simulink model "rfsoc4x2_ospfb_128"  (R2021a)
(part 2 of 339)

      mask prompts: Tile224_enable "Enable Tile"; t224_enable_mts "Enable Multi-Tile Sync"; t224_sample_rate "Sampling Rate (Msps)"; t224_clk_out "Clock Out (MHz)"; t224_enable_pll "Enable Tile PLLs"; t224_ref_clk "Reference Clock (MHz)"; t224_axi_stream_clk "Required AXI4-Stream Clock (MHz)"; t224_QT_adc0_enable "Enable ADC"; t224_QT_adc0_digital_output "Digital Output Data"; t224_QT_adc0_dec_mode "Decimation Mode"; t224_QT_adc0_sample_per_cycle "Samples per AXI4-Stream Cycle"; t224_QT_adc0_mixer_type "Mixer Type"; t224_QT_adc0_mixer_mode "Mixer Mode"; t224_QT_adc0_nco_freq "NCO Frequency (GHz)"; t224_QT_adc0_nco_phase "NCO Phase"; t224_QT_adc0_coarse_freq "Frequency"; t224_QT_adc0_nyquist_zone "Nyquist Zone"; t224_QT_adc0_cal_mode "Calibration Mode"; t224_QT_adc1_enable "Enable ADC"; t224_QT_adc1_digital_output "Digital Output Data"; t224_QT_adc1_dec_mode "Decimation Mode"; t224_QT_adc1_sample_per_cycle "Samples per AXI4-Stream Cycle"; t224_QT_adc1_mixer_type "Mixer Type"; t224_QT_adc1_mixer_mode "Mixer Mode"; t224_QT_adc1_nco_freq "NCO Frequency (GHz)"; t224_QT_adc1_nco_phase "NCO Phase"; t224_QT_adc1_coarse_freq "Frequency"; t224_QT_adc1_nyquist_zone "Nyquist Zone"; t224_QT_adc1_cal_mode "Calibration Mode"; t224_QT_adc2_enable "Enable ADC"; t224_QT_adc2_digital_output "Digital Output Data"; t224_QT_adc2_dec_mode "Decimation Mode"; t224_QT_adc2_sample_per_cycle "Samples per AXI4-Stream Cycle"; t224_QT_adc2_mixer_type "Mixer Type"; t224_QT_adc2_mixer_mode "Mixer Mode"; t224_QT_adc2_nco_freq "NCO Frequency (GHz)"; t224_QT_adc2_nco_phase "NCO Phase"; t224_QT_adc2_coarse_freq "Frequency"; t224_QT_adc2_nyquist_zone "Nyquist Zone"; t224_QT_adc2_cal_mode "Calibration Mode"; t224_QT_adc3_enable "Enable ADC"; t224_QT_adc3_digital_output "Digital Output Data"; t224_QT_adc3_dec_mode "Decimation Mode"; t224_QT_adc3_sample_per_cycle "Samples per AXI4-Stream Cycle"; t224_QT_adc3_mixer_type "Mixer Type"; t224_QT_adc3_mixer_mode "Mixer Mode"; t224_QT_adc3_nco_freq "NCO Frequency (GHz)"; t224_QT_adc3_nco_phase "NCO Phase"; t224_QT_adc3_coarse_freq "Frequency"; t224_QT_adc3_nyquist_zone "Nyquist Zone"; t224_QT_adc3_cal_mode "Calibration Mode"; t224_DT_adc0_enable "Enable ADC"; t224_DT_adc0_digital_output "Digital Output Data"; t224_DT_adc0_dec_mode "Decimation Mode"; t224_DT_adc0_sample_per_cycle "Samples per AXI4-Stream Cycle"; t224_DT_adc0_mixer_type "Mixer Type"; t224_DT_adc0_mixer_mode "Mixer Mode"; t224_DT_adc0_nco_freq "NCO Frequency (GHz)"; t224_DT_adc0_nco_phase "NCO Phase"; t224_DT_adc0_coarse_freq "Frequency"; t224_DT_adc0_nyquist_zone "Nyquist Zone"; t224_DT_adc0_cal_mode "Calibration Mode"; t224_DT_adc1_enable "Enable ADC"; t224_DT_adc1_digital_output "Digital Output Data"; t224_DT_adc1_dec_mode "Decimation Mode"; t224_DT_adc1_sample_per_cycle "Samples per AXI4-Stream Cycle"; t224_DT_adc1_mixer_type "Mixer Type"; t224_DT_adc1_mixer_mode "Mixer Mode"; t224_DT_adc1_nco_freq "NCO Frequency (GHz)"; t224_DT_adc1_nco_phase "NCO Phase"; t224_DT_adc1_coarse_freq "Frequency"; t224_DT_adc1_nyquist_zone "Nyquist Zone"; t224_DT_adc1_cal_mode "Calibration Mode"; Tile225_enable "Enable Tile"; t225_enable_mts "Enable Multi-Tile Sync"; t225_sample_rate "Sampling Rate (Msps)"; t225_clk_out "Clock Out (MHz)"; t225_enable_pll "Enable Tile PLLs"; t225_ref_clk "Reference Clock (MHz)"; t225_axi_stream_clk "Required AXI4-Stream Clock (MHz)"; t225_QT_adc0_enable "Enable ADC"; t225_QT_adc0_digital_output "Digital Output Data"; t225_QT_adc0_dec_mode "Decimation Mode"; t225_QT_adc0_sample_per_cycle "Samples per AXI4-Stream Cycle"; t225_QT_adc0_mixer_type "Mixer Type"; t225_QT_adc0_mixer_mode "Mixer Mode"; t225_QT_adc0_nco_freq "NCO Frequency (GHz)"; t225_QT_adc0_nco_phase "NCO Phase"; t225_QT_adc0_coarse_freq "Frequency"; t225_QT_adc0_nyquist_zone "Nyquist Zone"; t225_QT_adc0_cal_mode "Calibration Mode"; t225_QT_adc1_enable "Enable ADC"; t225_QT_adc1_digital_output "Digital Output Data"; t225_QT_adc1_dec_mode "Decimation Mode"; t225_QT_adc1_sample_per_cycle "Samples per AXI4-Stream Cycle"; t225_QT_adc1_mixer_type "Mixer Type"; t225_QT_adc1_mixer_mode "Mixer Mode"; t225_QT_adc1_nco_freq "NCO Frequency (GHz)"; t225_QT_adc1_nco_phase "NCO Phase"; t225_QT_adc1_coarse_freq "Frequency"; t225_QT_adc1_nyquist_zone "Nyquist Zone"; t225_QT_adc1_cal_mode "Calibration Mode"; t225_QT_adc2_enable "Enable ADC"; t225_QT_adc2_digital_output "Digital Output Data"; t225_QT_adc2_dec_mode "Decimation Mode"; t225_QT_adc2_sample_per_cycle "Samples per AXI4-Stream Cycle"; t225_QT_adc2_mixer_type "Mixer Type"; t225_QT_adc2_mixer_mode "Mixer Mode"; t225_QT_adc2_nco_freq "NCO Frequency (GHz)"; t225_QT_adc2_nco_phase "NCO Phase"; t225_QT_adc2_coarse_freq "Frequency"; t225_QT_adc2_nyquist_zone "Nyquist Zone"; t225_QT_adc2_cal_mode "Calibration Mode"; t225_QT_adc3_enable "Enable ADC"; t225_QT_adc3_digital_output "Digital Output Data"; t225_QT_adc3_dec_mode "Decimation Mode"; t225_QT_adc3_sample_per_cycle "Samples per AXI4-Stream Cycle"; t225_QT_adc3_mixer_type "Mixer Type"; t225_QT_adc3_mixer_mode "Mixer Mode"; t225_QT_adc3_nco_freq "NCO Frequency (GHz)"; t225_QT_adc3_nco_phase "NCO Phase"; t225_QT_adc3_coarse_freq "Frequency"; t225_QT_adc3_nyquist_zone "Nyquist Zone"; t225_QT_adc3_cal_mode "Calibration Mode"; t225_DT_adc0_enable "Enable ADC"; t225_DT_adc0_digital_output "Digital Output Data"; t225_DT_adc0_dec_mode "Decimation Mode"; t225_DT_adc0_sample_per_cycle "Samples per AXI4-Stream Cycle"; t225_DT_adc0_mixer_type "Mixer Type"; t225_DT_adc0_mixer_mode "Mixer Mode"; t225_DT_adc0_nco_freq "NCO Frequency (GHz)"; t225_DT_adc0_nco_phase "NCO Phase"; t225_DT_adc0_coarse_freq "Frequency"; t225_DT_adc0_nyquist_zone "Nyquist Zone"; t225_DT_adc0_cal_mode "Calibration Mode"; t225_DT_adc1_enable "Enable ADC"; t225_DT_adc1_digital_output "Digital Output Data"; t225_DT_adc1_dec_mode "Decimation Mode"; t225_DT_adc1_sample_per_cycle "Samples per AXI4-Stream Cycle"; t225_DT_adc1_mixer_type "Mixer Type"; t225_DT_adc1_mixer_mode "Mixer Mode"; t225_DT_adc1_nco_freq "NCO Frequency (GHz)"; t225_DT_adc1_nco_phase "NCO Phase"; t225_DT_adc1_coarse_freq "Frequency"; t225_DT_adc1_nyquist_zone "Nyquist Zone"; t225_DT_adc1_cal_mode "Calibration Mode"; Tile226_enable "Enable Tile"; t226_enable_mts "Enable Multi-Tile Sync"; t226_sample_rate "Sampling Rate (Msps)"; t226_clk_out "Clock Out (MHz)"; t226_enable_pll "Enable Tile PLLs"; t226_ref_clk "Reference Clock (MHz)"; t226_axi_stream_clk "Required AXI4-Stream Clock (MHz)"; t226_QT_adc0_enable "Enable ADC"; t226_QT_adc0_digital_output "Digital Output Data"; t226_QT_adc0_dec_mode "Decimation Mode"; t226_QT_adc0_sample_per_cycle "Samples per AXI4-Stream Cycle"; t226_QT_adc0_mixer_type "Mixer Type"; t226_QT_adc0_mixer_mode "Mixer Mode"; t226_QT_adc0_nco_freq "NCO Frequency (GHz)"; t226_QT_adc0_nco_phase "NCO Phase"; t226_QT_adc0_coarse_freq "Frequency"; t226_QT_adc0_nyquist_zone "Nyquist Zone"; t226_QT_adc0_cal_mode "Calibration Mode"; t226_QT_adc1_enable "Enable ADC"; t226_QT_adc1_digital_output "Digital Output Data"; t226_QT_adc1_dec_mode "Decimation Mode"; t226_QT_adc1_sample_per_cycle "Samples per AXI4-Stream Cycle"; t226_QT_adc1_mixer_type "Mixer Type"; t226_QT_adc1_mixer_mode "Mixer Mode"; t226_QT_adc1_nco_freq "NCO Frequency (GHz)"; t226_QT_adc1_nco_phase "NCO Phase"; t226_QT_adc1_coarse_freq "Frequency"; t226_QT_adc1_nyquist_zone "Nyquist Zone"; t226_QT_adc1_cal_mode "Calibration Mode"; t226_QT_adc2_enable "Enable ADC"; t226_QT_adc2_digital_output "Digital Output Data"; t226_QT_adc2_dec_mode "Decimation Mode"; t226_QT_adc2_sample_per_cycle "Samples per AXI4-Stream Cycle"; t226_QT_adc2_mixer_type "Mixer Type"; t226_QT_adc2_mixer_mode "Mixer Mode"; t226_QT_adc2_nco_freq "NCO Frequency (GHz)"; t226_QT_adc2_nco_phase "NCO Phase"; t226_QT_adc2_coarse_freq "Frequency"; t226_QT_adc2_nyquist_zone "Nyquist Zone"; t226_QT_adc2_cal_mode "Calibration Mode"; t226_QT_adc3_enable "Enable ADC"; t226_QT_adc3_digital_output "Digital Output Data"; t226_QT_adc3_dec_mode "Decimation Mode"; t226_QT_adc3_sample_per_cycle "Samples per AXI4-Stream Cycle"; t226_QT_adc3_mixer_type "Mixer Type"; t226_QT_adc3_mixer_mode "Mixer Mode"; t226_QT_adc3_nco_freq "NCO Frequency (GHz)"; t226_QT_adc3_nco_phase "NCO Phase"; t226_QT_adc3_coarse_freq "Frequency"; t226_QT_adc3_nyquist_zone "Nyquist Zone"; t226_QT_adc3_cal_mode "Calibration Mode"; t226_DT_adc0_enable "Enable ADC"; t226_DT_adc0_digital_output "Digital Output Data"; t226_DT_adc0_dec_mode "Decimation Mode"; t226_DT_adc0_sample_per_cycle "Samples per AXI4-Stream Cycle"; t226_DT_adc0_mixer_type "Mixer Type"; t226_DT_adc0_mixer_mode "Mixer Mode"; t226_DT_adc0_nco_freq "NCO Frequency (GHz)"; t226_DT_adc0_nco_phase "NCO Phase"; t226_DT_adc0_coarse_freq "Frequency"; t226_DT_adc0_nyquist_zone "Nyquist Zone"; t226_DT_adc0_cal_mode "Calibration Mode"; t226_DT_adc1_enable "Enable ADC"; t226_DT_adc1_digital_output "Digital Output Data"; t226_DT_adc1_dec_mode "Decimation Mode"; t226_DT_adc1_sample_per_cycle "Samples per AXI4-Stream Cycle"; t226_DT_adc1_mixer_type "Mixer Type"; t226_DT_adc1_mixer_mode "Mixer Mode"; t226_DT_adc1_nco_freq "NCO Frequency (GHz)"; t226_DT_adc1_nco_phase "NCO Phase"; t226_DT_adc1_coarse_freq "Frequency"; t226_DT_adc1_nyquist_zone "Nyquist Zone"; t226_DT_adc1_cal_mode "Calibration Mode"; Tile227_enable "Enable Tile"; t227_enable_mts "Enable Multi-Tile Sync"; t227_sample_rate "Sampling Rate (Msps)"; t227_clk_out "Clock Out (MHz)"; t227_enable_pll "Enable Tile PLLs"; t227_ref_clk "Reference Clock (MHz)"; t227_axi_stream_clk "Required AXI4-Stream Clock (MHz)"; t227_QT_adc0_enable "Enable ADC"; t227_QT_adc0_digital_output "Digital Output Data"; t227_QT_adc0_dec_mode "Decimation Mode"; t227_QT_adc0_sample_per_cycle "Samples per AXI4-Stream Cycle"; t227_QT_adc0_mixer_type "Mixer Type"; t227_QT_adc0_mixer_mode "Mixer Mode"; t227_QT_adc0_nco_freq "NCO Frequency (GHz)"; t227_QT_adc0_nco_phase "NCO Phase"; t227_QT_adc0_coarse_freq "Frequency"; t227_QT_adc0_nyquist_zone "Nyquist Zone"; t227_QT_adc0_cal_mode "Calibration Mode"; t227_QT_adc1_enable "Enable ADC"; t227_QT_adc1_digital_output "Digital Output Data"; t227_QT_adc1_dec_mode "Decimation Mode"; t227_QT_adc1_sample_per_cycle "Samples per AXI4-Stream Cycle"; t227_QT_adc1_mixer_type "Mixer Type"; t227_QT_adc1_mixer_mode "Mixer Mode"; t227_QT_adc1_nco_freq "NCO Frequency (GHz)"; t227_QT_adc1_nco_phase "NCO Phase"; t227_QT_adc1_coarse_freq "Frequency"; t227_QT_adc1_nyquist_zone "Nyquist Zone"; t227_QT_adc1_cal_mode "Calibration Mode"; t227_QT_adc2_enable "Enable ADC"; t227_QT_adc2_digital_output "Digital Output Data"; t227_QT_adc2_dec_mode "Decimation Mode"; t227_QT_adc2_sample_per_cycle "Samples per AXI4-Stream Cycle"; t227_QT_adc2_mixer_type "Mixer Type"; t227_QT_adc2_mixer_mode "Mixer Mode"; t227_QT_adc2_nco_freq "NCO Frequency (GHz)"; t227_QT_adc2_nco_phase "NCO Phase"; t227_QT_adc2_coarse_freq "Frequency"; t227_QT_adc2_nyquist_zone "Nyquist Zone"; t227_QT_adc2_cal_mode "Calibration Mode"; t227_QT_adc3_enable "Enable ADC"; t227_QT_adc3_digital_output "Digital Output Data"; t227_QT_adc3_dec_mode "Decimation Mode"; t227_QT_adc3_sample_per_cycle "Samples per AXI4-Stream Cycle"; t227_QT_adc3_mixer_type "Mixer Type"; t227_QT_adc3_mixer_mode "Mixer Mode"; t227_QT_adc3_nco_freq "NCO Frequency (GHz)"; t227_QT_adc3_nco_phase "NCO Phase"; t227_QT_adc3_coarse_freq "Frequency"; t227_QT_adc3_nyquist_zone "Nyquist Zone"; t227_QT_adc3_cal_mode "Calibration Mode"; t227_DT_adc0_enable "Enable ADC"; t227_DT_adc0_digital_output "Digital Output Data"; t227_DT_adc0_dec_mode "Decimation Mode"; t227_DT_adc0_sample_per_cycle "Samples per AXI4-Stream Cycle"; t227_DT_adc0_mixer_type "Mixer Type"; t227_DT_adc0_mixer_mode "Mixer Mode"; t227_DT_adc0_nco_freq "NCO Frequency (GHz)"; t227_DT_adc0_nco_phase "NCO Phase"; t227_DT_adc0_coarse_freq "Frequency"; t227_DT_adc0_nyquist_zone "Nyquist Zone"; t227_DT_adc0_cal_mode "Calibration Mode"; t227_DT_adc1_enable "Enable ADC"; t227_DT_adc1_digital_output "Digital Output Data"; t227_DT_adc1_dec_mode "Decimation Mode"; t227_DT_adc1_sample_per_cycle "Samples per AXI4-Stream Cycle"; t227_DT_adc1_mixer_type "Mixer Type"; t227_DT_adc1_mixer_mode "Mixer Mode"; t227_DT_adc1_nco_freq "NCO Frequency (GHz)"; t227_DT_adc1_nco_phase "NCO Phase"; t227_DT_adc1_coarse_freq "Frequency"; t227_DT_adc1_nyquist_zone "Nyquist Zone"; t227_DT_adc1_cal_mode "Calibration Mode"; Tile228_enable "Enable Tile"; t228_enable_mts "Enable Multi-Tile Sync"; t228_sample_rate "Sampling Rate (Msps)"; t228_clk_out "Clock Out (MHz)"; t228_enable_pll "Enable Tile PLLs"; t228_ref_clk "Reference Clock (MHz)"; t228_axi_stream_clk "Required AXI4-Stream Clock (MHz)"; t228_output_power "Output Power"; t228_QT_dac0_enable "Enable DAC"; t228_QT_dac0_analog_output "Analog Output Data"; t228_QT_dac0_inter_mode "Interpolation Mode"; t228_QT_dac0_sample_per_cycle "Samples per AXI4-Stream Cycle"; t228_QT_dac0_datapath_mode "Datapath Mode"; t228_QT_dac0_mixer_type "Mixer Type"; t228_QT_dac0_mixer_mode "Mixer Mode"; t228_QT_dac0_nco_freq "NCO Frequency (GHz)"; t228_QT_dac0_nco_phase "NCO Phase"; t228_QT_dac0_coarse_freq "Frequency"; t228_QT_dac0_nyquist_zone "Nyquist Zone"; t228_QT_dac0_decode_mode "Decoder Mode"; t228_QT_dac1_enable "Enable DAC"; t228_QT_dac1_analog_output "Analog Output Data"; t228_QT_dac1_inter_mode "Interpolation Mode"; t228_QT_dac1_sample_per_cycle "Samples per AXI4-Stream Cycle"; t228_QT_dac1_datapath_mode "Datapath Mode"; t228_QT_dac1_mixer_type "Mixer Type"; t228_QT_dac1_mixer_mode "Mixer Mode"; t228_QT_dac1_nco_freq "NCO Frequency (GHz)"; t228_QT_dac1_nco_phase "NCO Phase"; t228_QT_dac1_coarse_freq "Frequency"; t228_QT_dac1_nyquist_zone "Nyquist Zone"; t228_QT_dac1_decode_mode "Decoder Mode"; t228_QT_dac2_enable "Enable DAC"; t228_QT_dac2_analog_output "Analog Output Data"; t228_QT_dac2_inter_mode "Interpolation Mode"; t228_QT_dac2_sample_per_cycle "Samples per AXI4-Stream Cycle"; t228_QT_dac2_datapath_mode "Datapath Mode"; t228_QT_dac2_mixer_type "Mixer Type"; t228_QT_dac2_mixer_mode "Mixer Mode"; t228_QT_dac2_nco_freq "NCO Frequency (GHz)"; t228_QT_dac2_nco_phase "NCO Phase"; t228_QT_dac2_coarse_freq "Frequency"; t228_QT_dac2_nyquist_zone "Nyquist Zone"; t228_QT_dac2_decode_mode "Decoder Mode"; t228_QT_dac3_enable "Enable DAC"; t228_QT_dac3_analog_output "Analog Output Data"; t228_QT_dac3_inter_mode "Interpolation Mode"; t228_QT_dac3_sample_per_cycle "Samples per AXI4-Stream Cycle"; t228_QT_dac3_datapath_mode "Datapath Mode"; t228_QT_dac3_mixer_type "Mixer Type"; t228_QT_dac3_mixer_mode "Mixer Mode"; t228_QT_dac3_nco_freq "NCO Frequency (GHz)"; t228_QT_dac3_nco_phase "NCO Phase"; t228_QT_dac3_coarse_freq "Frequency"; t228_QT_dac3_nyquist_zone "Nyquist Zone"; t228_QT_dac3_decode_mode "Decoder Mode"; t228_DT_dac0_enable "Enable DAC"; t228_DT_dac0_analog_output "Analog Output Data"; t228_DT_dac0_inter_mode "Interpolation Mode"; t228_DT_dac0_sample_per_cycle "Samples per AXI4-Stream Cycle"; t228_DT_dac0_mixer_type "Mixer Type"; t228_DT_dac0_mixer_mode "Mixer Mode"; t228_DT_dac0_nco_freq "NCO Frequency (GHz)"; t228_DT_dac0_nco_phase "NCO Phase"; t228_DT_dac0_coarse_freq "Frequency"; t228_DT_dac0_nyquist_zone "Nyquist Zone"; t228_DT_dac0_decode_mode "Decoder Mode"; t228_DT_dac1_enable "Enable DAC"; t228_DT_dac1_analog_output "Analog Output Data"; t228_DT_dac1_inter_mode "Interpolation Mode"; t228_DT_dac1_sample_per_cycle "Samples per AXI4-Stream Cycle"; t228_DT_dac1_mixer_type "Mixer Type"; t228_DT_dac1_mixer_mode "Mixer Mode"; t228_DT_dac1_nco_freq "NCO Frequency (GHz)"; t228_DT_dac1_nco_phase "NCO Phase"; t228_DT_dac1_coarse_freq "Frequency"; t228_DT_dac1_nyquist_zone "Nyquist Zone"; t228_DT_dac1_decode_mode "Decoder Mode"; Tile229_enable "Enable Tile"; t229_enable_mts "Enable Multi-Tile Sync"; t229_sample_rate "Sampling Rate (Msps)"; t229_clk_out "Clock Out (MHz)"; t229_enable_pll "Enable Tile PLLs"; t229_ref_clk "Reference Clock (MHz)"; t229_axi_stream_clk "Required AXI4-Stream Clock (MHz)"; t229_output_power "Output Power"; t229_QT_dac0_enable "Enable DAC"; t229_QT_dac0_analog_output "Analog Output Data"; t229_QT_dac0_inter_mode "Interpolation Mode"; t229_QT_dac0_sample_per_cycle "Samples per AXI4-Stream Cycle"; t229_QT_dac0_datapath_mode "Datapath Mode"; t229_QT_dac0_mixer_type "Mixer Type"; t229_QT_dac0_mixer_mode "Mixer Mode"; t229_QT_dac0_nco_freq "NCO Frequency (GHz)"; t229_QT_dac0_nco_phase "NCO Phase"; t229_QT_dac0_coarse_freq "Frequency"; t229_QT_dac0_nyquist_zone "Nyquist Zone"; t229_QT_dac0_decode_mode "Decoder Mode"; t229_QT_dac1_enable "Enable DAC"; t229_QT_dac1_analog_output "Analog Output Data"; t229_QT_dac1_inter_mode "Interpolation Mode"; t229_QT_dac1_sample_per_cycle "Samples per AXI4-Stream Cycle"; t229_QT_dac1_datapath_mode "Datapath Mode"; t229_QT_dac1_mixer_type "Mixer Type"; t229_QT_dac1_mixer_mode "Mixer Mode"; t229_QT_dac1_nco_freq "NCO Frequency (GHz)"; t229_QT_dac1_nco_phase "NCO Phase"; t229_QT_dac1_coarse_freq "Frequency"; t229_QT_dac1_nyquist_zone "Nyquist Zone"; t229_QT_dac1_decode_mode "Decoder Mode"; t229_QT_dac2_enable "Enable DAC"; t229_QT_dac2_analog_output "Analog Output Data"; t229_QT_dac2_inter_mode "Interpolation Mode"; t229_QT_dac2_sample_per_cycle "Samples per AXI4-Stream Cycle"; t229_QT_dac2_datapath_mode "Datapath Mode"; t229_QT_dac2_mixer_type "Mixer Type"; t229_QT_dac2_mixer_mode "Mixer Mode"; t229_QT_dac2_nco_freq "NCO Frequency (GHz)"; t229_QT_dac2_nco_phase "NCO Phase"; t229_QT_dac2_coarse_freq "Frequency"; t229_QT_dac2_nyquist_zone "Nyquist Zone"; t229_QT_dac2_decode_mode "Decoder Mode"; t229_QT_dac3_enable "Enable DAC"; t229_QT_dac3_analog_output "Analog Output Data"; t229_QT_dac3_inter_mode "Interpolation Mode"; t229_QT_dac3_sample_per_cycle "Samples per AXI4-Stream Cycle"; t229_QT_dac3_datapath_mode "Datapath Mode"; t229_QT_dac3_mixer_type "Mixer Type"; t229_QT_dac3_mixer_mode "Mixer Mode"; t229_QT_dac3_nco_freq "NCO Frequency (GHz)"; t229_QT_dac3_nco_phase "NCO Phase"; t229_QT_dac3_coarse_freq "Frequency"; t229_QT_dac3_nyquist_zone "Nyquist Zone"; t229_QT_dac3_decode_mode "Decoder Mode"; t229_DT_dac0_enable "Enable DAC"; t229_DT_dac0_analog_output "Analog Output Data"; t229_DT_dac0_inter_mode "Interpolation Mode"; t229_DT_dac0_sample_per_cycle "Samples per AXI4-Stream Cycle"; t229_DT_dac0_mixer_type "Mixer Type"; t229_DT_dac0_mixer_mode "Mixer Mode"; t229_DT_dac0_nco_freq "NCO Frequency (GHz)"; t229_DT_dac0_nco_phase "NCO Phase"; t229_DT_dac0_coarse_freq "Frequency"; t229_DT_dac0_nyquist_zone "Nyquist Zone"; t229_DT_dac0_decode_mode "Decoder Mode"; t229_DT_dac1_enable "Enable DAC"; t229_DT_dac1_analog_output "Analog Output Data"; t229_DT_dac1_inter_mode "Interpolation Mode"; t229_DT_dac1_sample_per_cycle "Samples per AXI4-Stream Cycle"; t229_DT_dac1_mixer_type "Mixer Type"; t229_DT_dac1_mixer_mode "Mixer Mode"; t229_DT_dac1_nco_freq "NCO Frequency (GHz)"; t229_DT_dac1_nco_phase "NCO Phase"; t229_DT_dac1_coarse_freq "Frequency"; t229_DT_dac1_nyquist_zone "Nyquist Zone"; t229_DT_dac1_decode_mode "Decoder Mode"; Tile230_enable "Enable Tile"; t230_enable_mts "Enable Multi-Tile Sync"; t230_sample_rate "Sampling Rate (Msps)"; t230_clk_out "Clock Out (MHz)"; t230_enable_pll "Enable Tile PLLs"; t230_ref_clk "Reference Clock (MHz)"; t230_axi_stream_clk "Required AXI4-Stream Clock (MHz)"; t230_output_power "Output Power"; t230_QT_dac0_enable "Enable DAC"; t230_QT_dac0_analog_output "Analog Output Data"; t230_QT_dac0_inter_mode "Interpolation Mode"; t230_QT_dac0_sample_per_cycle "Samples per AXI4-Stream Cycle"; t230_QT_dac0_datapath_mode "Datapath Mode"; t230_QT_dac0_mixer_type "Mixer Type"; t230_QT_dac0_mixer_mode "Mixer Mode"; t230_QT_dac0_nco_freq "NCO Frequency (GHz)"; t230_QT_dac0_nco_phase "NCO Phase"; t230_QT_dac0_coarse_freq "Frequency"; t230_QT_dac0_nyquist_zone "Nyquist Zone"; t230_QT_dac0_decode_mode "Decoder Mode"; t230_QT_dac1_enable "Enable DAC"; t230_QT_dac1_analog_output "Analog Output Data"; t230_QT_dac1_inter_mode "Interpolation Mode"; t230_QT_dac1_sample_per_cycle "Samples per AXI4-Stream Cycle"; t230_QT_dac1_datapath_mode "Datapath Mode"; t230_QT_dac1_mixer_type "Mixer Type"; t230_QT_dac1_mixer_mode "Mixer Mode"; t230_QT_dac1_nco_freq "NCO Frequency (GHz)"; t230_QT_dac1_nco_phase "NCO Phase"; t230_QT_dac1_coarse_freq "Frequency"; t230_QT_dac1_nyquist_zone "Nyquist Zone"; t230_QT_dac1_decode_mode "Decoder Mode"; t230_QT_dac2_enable "Enable DAC"; t230_QT_dac2_analog_output "Analog Output Data"; t230_QT_dac2_inter_mode "Interpolation Mode"; t230_QT_dac2_sample_per_cycle "Samples per AXI4-Stream Cycle"; t230_QT_dac2_datapath_mode "Datapath Mode"; t230_QT_dac2_mixer_type "Mixer Type"; t230_QT_dac2_mixer_mode "Mixer Mode"; t230_QT_dac2_nco_freq "NCO Frequency (GHz)"; t230_QT_dac2_nco_phase "NCO Phase"; t230_QT_dac2_coarse_freq "Frequency"; t230_QT_dac2_nyquist_zone "Nyquist Zone"; t230_QT_dac2_decode_mode "Decoder Mode"; t230_QT_dac3_enable "Enable DAC"; t230_QT_dac3_analog_output "Analog Output Data"; t230_QT_dac3_inter_mode "Interpolation Mode"; t230_QT_dac3_sample_per_cycle "Samples per AXI4-Stream Cycle"; t230_QT_dac3_datapath_mode "Datapath Mode"; t230_QT_dac3_mixer_type "Mixer Type"; t230_QT_dac3_mixer_mode "Mixer Mode"; t230_QT_dac3_nco_freq "NCO Frequency (GHz)"; t230_QT_dac3_nco_phase "NCO Phase"; t230_QT_dac3_coarse_freq "Frequency"; t230_QT_dac3_nyquist_zone "Nyquist Zone"; t230_QT_dac3_decode_mode "Decoder Mode"; t230_DT_dac0_enable "Enable DAC"; t230_DT_dac0_analog_output "Analog Output Data"; t230_DT_dac0_inter_mode "Interpolation Mode"; t230_DT_dac0_sample_per_cycle "Samples per AXI4-Stream Cycle"; t230_DT_dac0_mixer_type "Mixer Type"; t230_DT_dac0_mixer_mode "Mixer Mode"; t230_DT_dac0_nco_freq "NCO Frequency (GHz)"; t230_DT_dac0_nco_phase "NCO Phase"; t230_DT_dac0_coarse_freq "Frequency"; t230_DT_dac0_nyquist_zone "Nyquist Zone"; t230_DT_dac0_decode_mode "Decoder Mode"; t230_DT_dac1_enable "Enable DAC"; t230_DT_dac1_analog_output "Analog Output Data"; t230_DT_dac1_inter_mode "Interpolation Mode"; t230_DT_dac1_sample_per_cycle "Samples per AXI4-Stream Cycle"; t230_DT_dac1_mixer_type "Mixer Type"; t230_DT_dac1_mixer_mode "Mixer Mode"; t230_DT_dac1_nco_freq "NCO Frequency (GHz)"; t230_DT_dac1_nco_phase "NCO Phase"; t230_DT_dac1_coarse_freq "Frequency"; t230_DT_dac1_nyquist_zone "Nyquist Zone"; t230_DT_dac1_decode_mode "Decoder Mode"; Tile231_enable "Enable Tile"; t231_enable_mts "Enable Multi-Tile Sync"; t231_sample_rate "Sampling Rate (Msps)"; t231_clk_out "Clock Out (MHz)"; t231_enable_pll "Enable Tile PLLs"; t231_ref_clk "Reference Clock (MHz)"; t231_axi_stream_clk "Required AXI4-Stream Clock (MHz)"; t231_output_power "Output Power"; t231_QT_dac0_enable "Enable DAC"; t231_QT_dac0_analog_output "Analog Output Data"; t231_QT_dac0_inter_mode "Interpolation Mode"; t231_QT_dac0_sample_per_cycle "Samples per AXI4-Stream Cycle"; t231_QT_dac0_datapath_mode "Datapath Mode"; t231_QT_dac0_mixer_type "Mixer Type"; t231_QT_dac0_mixer_mode "Mixer Mode"; t231_QT_dac0_nco_freq "NCO Frequency (GHz)"; t231_QT_dac0_nco_phase "NCO Phase"; t231_QT_dac0_coarse_freq "Frequency"; t231_QT_dac0_nyquist_zone "Nyquist Zone"; t231_QT_dac0_decode_mode "Decoder Mode"; t231_QT_dac1_enable "Enable DAC"; t231_QT_dac1_analog_output "Analog Output Data"; t231_QT_dac1_inter_mode "Interpolation Mode"; t231_QT_dac1_sample_per_cycle "Samples per AXI4-Stream Cycle"; t231_QT_dac1_datapath_mode "Datapath Mode"; t231_QT_dac1_mixer_type "Mixer Type"; t231_QT_dac1_mixer_mode "Mixer Mode"; t231_QT_dac1_nco_freq "NCO Frequency (GHz)"; t231_QT_dac1_nco_phase "NCO Phase"; t231_QT_dac1_coarse_freq "Frequency"; t231_QT_dac1_nyquist_zone "Nyquist Zone"; t231_QT_dac1_decode_mode "Decoder Mode"; t231_QT_dac2_enable "Enable DAC"; t231_QT_dac2_analog_output "Analog Output Data"; t231_QT_dac2_inter_mode "Interpolation Mode"; t231_QT_dac2_sample_per_cycle "Samples per AXI4-Stream Cycle"; t231_QT_dac2_datapath_mode "Datapath Mode"; t231_QT_dac2_mixer_type "Mixer Type"; t231_QT_dac2_mixer_mode "Mixer Mode"; t231_QT_dac2_nco_freq "NCO Frequency (GHz)"; t231_QT_dac2_nco_phase "NCO Phase"; t231_QT_dac2_coarse_freq "Frequency"; t231_QT_dac2_nyquist_zone "Nyquist Zone"; t231_QT_dac2_decode_mode "Decoder Mode"; t231_QT_dac3_enable "Enable DAC"; t231_QT_dac3_analog_output "Analog Output Data"; t231_QT_dac3_inter_mode "Interpolation Mode"; t231_QT_dac3_sample_per_cycle "Samples per AXI4-Stream Cycle"; t231_QT_dac3_datapath_mode "Datapath Mode"; t231_QT_dac3_mixer_type "Mixer Type"; t231_QT_dac3_mixer_mode "Mixer Mode"; t231_QT_dac3_nco_freq "NCO Frequency (GHz)"; t231_QT_dac3_nco_phase "NCO Phase"; t231_QT_dac3_coarse_freq "Frequency"; t231_QT_dac3_nyquist_zone "Nyquist Zone"; t231_QT_dac3_decode_mode "Decoder Mode"; t231_DT_dac0_enable "Enable DAC"; t231_DT_dac0_analog_output "Analog Output Data"; t231_DT_dac0_inter_mode "Interpolation Mode"; t231_DT_dac0_sample_per_cycle "Samples per AXI4-Stream Cycle"; t231_DT_dac0_mixer_type "Mixer Type"; t231_DT_dac0_mixer_mode "Mixer Mode"; t231_DT_dac0_nco_freq "NCO Frequency (GHz)"; t231_DT_dac0_nco_phase "NCO Phase"; t231_DT_dac0_coarse_freq "Frequency"; t231_DT_dac0_nyquist_zone "Nyquist Zone"; t231_DT_dac0_decode_mode "Decoder Mode"; t231_DT_dac1_enable "Enable DAC"; t231_DT_dac1_analog_output "Analog Output Data"; t231_DT_dac1_inter_mode "Interpolation Mode"; t231_DT_dac1_sample_per_cycle "Samples per AXI4-Stream Cycle"; t231_DT_dac1_mixer_type "Mixer Type"; t231_DT_dac1_mixer_mode "Mixer Mode"; t231_DT_dac1_nco_freq "NCO Frequency (GHz)"; t231_DT_dac1_nco_phase "NCO Phase"; t231_DT_dac1_coarse_freq "Frequency"; t231_DT_dac1_nyquist_zone "Nyquist Zone"; t231_DT_dac1_decode_mode "Decoder Mode"; t224_has_adc_clk "Has Clock"; t224_adc_clk_src "Clock Source Tile"; t224_clk_dist "Distribute Clock"; t225_has_adc_clk "Has Clock"; t225_adc_clk_src "Clock Source Tile"; t225_clk_dist "Distribute Clock"; t226_has_adc_clk "Has Clock"; t226_adc_clk_src "Clock Source Tile"; t226_clk_dist "Distribute Clock"; t227_has_adc_clk "Has Clock"; t227_adc_clk_src "Clock Source Tile"; t227_clk_dist "Distribute Clock"; t228_has_dac_clk "Has Clock"; t228_dac_clk_src "Clock Source Tile"; t228_clk_dist "Distribute Clock"; t229_has_dac_clk "Has Clock"; t229_dac_clk_src "Clock Source Tile"; t229_clk_dist "Distribute Clock"; t230_has_dac_clk "Has Clock"; t230_dac_clk_src "Clock Source Tile"; t230_clk_dist "Distribute Clock"; t231_has_dac_clk "Has Clock"; t231_dac_clk_src "Clock Source Tile"; t231_clk_dist "Distribute Clock"
      mask help: CASPER RFDC
      mask init:
      | if chk_param(gcb,'runinit','1')
      |     if chk_param(gcb,'forceredraw','0')
      |         rfdc_mask(gcb,0);
      |     else
      |         rfdc_mask(gcb,1);
      |         set_param(gcb,'forceredraw','0')
      |     end
      |     if chk_param(gcb,'maskopening','1')
      |         set_param(gcb,'runinit','0')
      |     end
      | end
      mask Help: eval('xlWeb([getenv(''MLIB_ROOT''), ''\doc\html\adc_zcu111\adc_zcu111.html''])')
      mask Callback maskopening:
      | %assignin('base','mask_opening',1)
      | %assignin('base','run_init',1)
      | set_param(gcb,'maskopening','1')
      mask Callback runinit: set_param(gcb,'runinit','1')
      mask Callback Tile224_enable: enable_mts_opt(gcb);
      mask Callback t224_sample_rate: update_rfdc_clocking(gcb,224);
      mask TypeOptions t224_clk_out: 150 | 75 | 37.5 | 18.75
      mask Callback t224_enable_pll:
      | %update_rfdc_clocking(gcb);
      | update_pll(gcb,224);
      mask TypeOptions t224_ref_clk: 738.462 | 685.714 | 640 | 600 | 564.706 | 533.333 | 505.263 | 480 | 457.143 | 436.364 | 417.391 | 400 | 384 | 369.231 | 355.556 | 342.857 | 331.034 | 320 | 309.677 | 300 | 290.909 | 282.353 | 274.286 | 266.667 | 259.459 | 252.632 | 246.154 | 240 | 234.146 | 228.571 | 223.256 | 218.182 | 213.333 | 208.696 | 204.255 | 200 | 195.918 | 192 | 188.235 | 184.615 | 181.132 | 177.778 | 174.545 | 171.429 | 168.421 | 165.517 | 162.712 | 160 | 157.377 | 154.839 | 152.381 | 150 | 147.692 | 145.455 | 143.284 | 141.176 | 139.13 | 137.143 | 135.211 | 133.333 | 131.507 | 129.73 | 128 | 126.316 | 124.675 | 123.077 | 121.519 | 120 | 118.519 | 117.073 | 115.663 | 114.286 | 112.941 | 111.628 | 110.345 | 109.091 | 107.865 | 106.667 | 105.495 | 104.348 | 103.226
      mask Callback t224_QT_adc0_enable: enable_adc_opt(gcb,224,0,'QT');
      mask TypeOptions t224_QT_adc0_digital_output: Real | I/Q
      mask Callback t224_QT_adc0_digital_output:
      | validate_digital_data(gcb,224,0,'QT');
      | update_axis_clk(gcb,224);
      mask TypeOptions t224_QT_adc0_dec_mode: 1x | 2x | 3x | 4x | 5x | 6x | 8x | 10x | 12x | 16x | 20x | 24x | 40x
      mask Callback t224_QT_adc0_dec_mode:
      | % if I/Q output mode, need to copy interp factor before updating axis clk
      | % note only the even slice for the tile makes this check
      | if chk_param(gcb, 't224_QT_adc0_mixer_mode', 'I/Q -> I/Q')
      |   dec_mode = get_param(gcb, 't224_QT_adc0_dec_mode');
      |   set_param(gcb, 't224_QT_adc1_dec_mode', dec_mode);
      | end
      | 
      | update_axis_clk(gcb,224);
      mask TypeOptions t224_QT_adc0_sample_per_cycle: 4 | 5 | 6 | 7 | 8 | 9 | 10 | 11 | 12
      mask Callback t224_QT_adc0_sample_per_cycle:
      | % if I/Q output mode, need to copy samples per clk before updating axis clk
      | % note only the even slice for the tile makes this check
      | if chk_param(gcb, 't224_QT_adc0_mixer_mode', 'I/Q -> I/Q')
      |   spc = get_param(gcb, 't224_QT_adc0_sample_per_cycle');
      |   set_param(gcb, 't224_QT_adc1_sample_per_cycle', spc);
      | end
      | update_axis_clk_label(gcb,224);
      mask TypeOptions t224_QT_adc0_mixer_type: Bypassed
      mask Callback t224_QT_adc0_mixer_type: mixertype_callback(gcb,224,0,'QT');
      mask TypeOptions t224_QT_adc0_mixer_mode: Real -> Real
      mask Callback t224_QT_adc0_mixer_mode: mixer_callback(gcb,224,0,'QT');
      mask TypeOptions t224_QT_adc0_coarse_freq: 0
      mask TypeOptions t224_QT_adc0_nyquist_zone: Zone 1 | Zone 2
      mask TypeOptions t224_QT_adc0_cal_mode: Mode 1 | Mode 2
      mask Callback t224_QT_adc1_enable: enable_adc_opt(gcb,224,1,'QT');
      mask TypeOptions t224_QT_adc1_digital_output: Real | I/Q
      mask Callback t224_QT_adc1_digital_output:
      | validate_digital_data(gcb,224,1,'QT');
      | update_axis_clk(gcb,224);
      mask TypeOptions t224_QT_adc1_dec_mode: 1x | 2x | 3x | 4x | 5x | 6x | 8x | 10x | 12x | 16x | 20x | 24x | 40x
      mask Callback t224_QT_adc1_dec_mode: update_axis_clk(gcb,224);
      mask TypeOptions t224_QT_adc1_sample_per_cycle: 4 | 5 | 6 | 7 | 8 | 9 | 10 | 11 | 12
      mask Callback t224_QT_adc1_sample_per_cycle: update_axis_clk_label(gcb,224);
      mask TypeOptions t224_QT_adc1_mixer_type: Bypassed
      mask Callback t224_QT_adc1_mixer_type: mixertype_callback(gcb,224,1,'QT');
      mask TypeOptions t224_QT_adc1_mixer_mode: Real -> Real
      mask Callback t224_QT_adc1_mixer_mode: mixer_callback(gcb,224,1,'QT')
      mask TypeOptions t224_QT_adc1_coarse_freq: 0
      mask TypeOptions t224_QT_adc1_nyquist_zone: Zone 1 | Zone 2
      mask TypeOptions t224_QT_adc1_cal_mode: Mode 1 | Mode 2
      mask Callback t224_QT_adc2_enable: enable_adc_opt(gcb,224,2,'QT');
      mask TypeOptions t224_QT_adc2_digital_output: Real | I/Q
      mask Callback t224_QT_adc2_digital_output:
      | validate_digital_data(gcb,224,2,'QT');
      | update_axis_clk(gcb,224);
      mask TypeOptions t224_QT_adc2_dec_mode: 1x | 2x | 3x | 4x | 5x | 6x | 8x | 10x | 12x | 16x | 20x | 24x | 40x
      mask Callback t224_QT_adc2_dec_mode:
      | % if I/Q output mode, need to copy interp factor before updating axis clk
      | % note only the even slice for the tile makes this check
      | if chk_param(gcb, 't224_QT_adc2_mixer_mode', 'I/Q -> I/Q')
      |   dec_mode = get_param(gcb, 't224_QT_adc2_dec_mode');
      |   set_param(gcb, 't224_QT_adc3_dec_mode', dec_mode);
      | end
      | update_axis_clk(gcb,224);
      mask TypeOptions t224_QT_adc2_sample_per_cycle: 4 | 5 | 6 | 7 | 8 | 9 | 10 | 11 | 12
      mask Callback t224_QT_adc2_sample_per_cycle:
      | % if I/Q output mode, need to copy samples per clk before updating axis clk
      | % note only the even slice for the tile makes this check
      | if chk_param(gcb, 't224_QT_adc2_mixer_mode', 'I/Q -> I/Q')
      |   spc = get_param(gcb, 't224_QT_adc2_sample_per_cycle');
      |   set_param(gcb, 't224_QT_adc3_sample_per_cycle', spc);
      | end
      | update_axis_clk_label(gcb,224);
      mask TypeOptions t224_QT_adc2_mixer_type: Bypassed
      mask Callback t224_QT_adc2_mixer_type: mixertype_callback(gcb,224,2,'QT');
      mask TypeOptions t224_QT_adc2_mixer_mode: Real -> Real
      mask Callback t224_QT_adc2_mixer_mode: mixer_callback(gcb,224,2,'QT')
      mask TypeOptions t224_QT_adc2_coarse_freq: 0
      mask TypeOptions t224_QT_adc2_nyquist_zone: Zone 1 | Zone 2
      mask TypeOptions t224_QT_adc2_cal_mode: Mode 1 | Mode 2
      mask Callback t224_QT_adc3_enable: enable_adc_opt(gcb,224,3,'QT');
      mask TypeOptions t224_QT_adc3_digital_output: Real | I/Q
      mask Callback t224_QT_adc3_digital_output:
      | validate_digital_data(gcb,224,3,'QT');
      | update_axis_clk(gcb,224);
      mask TypeOptions t224_QT_adc3_dec_mode: 1x | 2x | 3x | 4x | 5x | 6x | 8x | 10x | 12x | 16x | 20x | 24x | 40x
      mask Callback t224_QT_adc3_dec_mode: update_axis_clk(gcb,224);
      mask TypeOptions t224_QT_adc3_sample_per_cycle: 4 | 5 | 6 | 7 | 8 | 9 | 10 | 11 | 12
      mask Callback t224_QT_adc3_sample_per_cycle: update_axis_clk_label(gcb,224);
      mask TypeOptions t224_QT_adc3_mixer_type: Bypassed
      mask Callback t224_QT_adc3_mixer_type: mixertype_callback(gcb,224,3,'QT');
      mask TypeOptions t224_QT_adc3_mixer_mode: Real -> Real
      mask Callback t224_QT_adc3_mixer_mode: mixer_callback(gcb,224,3,'QT')
      mask TypeOptions t224_QT_adc3_coarse_freq: 0
      mask TypeOptions t224_QT_adc3_nyquist_zone: Zone 1 | Zone 2
      mask TypeOptions t224_QT_adc3_cal_mode: Mode 1 | Mode 2
      mask Callback t224_DT_adc0_enable: enable_adc_opt(gcb,224,0,'DT');
      mask TypeOptions t224_DT_adc0_digital_output: Real | I/Q
      mask Callback t224_DT_adc0_digital_output:
      | validate_digital_data(gcb,224,0,'DT');
      | update_axis_clk(gcb,224);
      mask TypeOptions t224_DT_adc0_dec_mode: 1x | 2x | 3x | 4x | 5x | 6x | 8x | 10x | 12x | 16x | 20x | 24x | 40x
      mask Callback t224_DT_adc0_dec_mode:
      | % if I/Q output mode, need to copy interp factor before updating axis clk
      | % note only the even slice for the tile makes this check
      | if chk_param(gcb, 't224_DT_adc0_mixer_mode', 'I/Q -> I/Q')
      |   dec_mode = get_param(gcb, 't224_DT_adc0_dec_mode');
      |   set_param(gcb, 't224_DT_adc1_dec_mode', dec_mode);
      | end
      | 
      | update_axis_clk(gcb,224);
      mask TypeOptions t224_DT_adc0_sample_per_cycle: 5 | 6 | 7 | 8 | 9 | 10 | 11 | 12
      mask Callback t224_DT_adc0_sample_per_cycle:
      | % if I/Q output mode, need to copy samples per clk before updating axis clk
      | % note only the even slice for the tile makes this check
      | if chk_param(gcb, 't224_DT_adc0_mixer_mode', 'I/Q -> I/Q')
      |   spc = get_param(gcb, 't224_DT_adc0_sample_per_cycle');
      |   set_param(gcb, 't224_DT_adc1_sample_per_cycle', spc);
      | end
      | update_axis_clk_label(gcb,224);
      mask TypeOptions t224_DT_adc0_mixer_type: Bypassed
      mask Callback t224_DT_adc0_mixer_type: mixertype_callback(gcb,224,0,'DT');
      mask TypeOptions t224_DT_adc0_mixer_mode: Real -> Real
      mask Callback t224_DT_adc0_mixer_mode: mixer_callback(gcb,224,0,'DT');
      mask TypeOptions t224_DT_adc0_coarse_freq: 0
      mask TypeOptions t224_DT_adc0_nyquist_zone: Zone 1 | Zone 2
      mask TypeOptions t224_DT_adc0_cal_mode: Mode 1 | Mode 2
      mask Callback t224_DT_adc1_enable: enable_adc_opt(gcb,224,1,'DT');
      mask TypeOptions t224_DT_adc1_digital_output: Real | I/Q
      mask Callback t224_DT_adc1_digital_output:
      | validate_digital_data(gcb,224,1,'DT');
      | update_axis_clk(gcb,224);
      mask TypeOptions t224_DT_adc1_dec_mode: 1x | 2x | 3x | 4x | 5x | 6x | 8x | 10x | 12x | 16x | 20x | 24x | 40x
      mask Callback t224_DT_adc1_dec_mode: update_axis_clk(gcb,224);
      mask TypeOptions t224_DT_adc1_sample_per_cycle: 5 | 6 | 7 | 8 | 9 | 10 | 11 | 12
      mask Callback t224_DT_adc1_sample_per_cycle:
      | %update_axis_clk(gcb);
      | update_axis_clk_label(gcb,224);
      mask TypeOptions t224_DT_adc1_mixer_type: Bypassed
      mask Callback t224_DT_adc1_mixer_type: mixertype_callback(gcb,224,1,'DT');
      mask TypeOptions t224_DT_adc1_mixer_mode: Real -> Real
      mask Callback t224_DT_adc1_mixer_mode: mixer_callback(gcb,224,1,'DT');
      mask TypeOptions t224_DT_adc1_coarse_freq: 0
      mask TypeOptions t224_DT_adc1_nyquist_zone: Zone 1 | Zone 2
      mask TypeOptions t224_DT_adc1_cal_mode: Mode 1 | Mode 2
      mask Callback t225_sample_rate: update_rfdc_clocking(gcb,225);
      mask TypeOptions t225_clk_out: 150 | 75 | 37.5 | 18.75
      mask Callback t225_enable_pll:
      | %update_rfdc_clocking(gcb);
      | update_pll(gcb,225);
      mask TypeOptions t225_ref_clk: 738.462 | 685.714 | 640 | 600 | 564.706 | 533.333 | 505.263 | 480 | 457.143 | 436.364 | 417.391 | 400 | 384 | 369.231 | 355.556 | 342.857 | 331.034 | 320 | 309.677 | 300 | 290.909 | 282.353 | 274.286 | 266.667 | 259.459 | 252.632 | 246.154 | 240 | 234.146 | 228.571 | 223.256 | 218.182 | 213.333 | 208.696 | 204.255 | 200 | 195.918 | 192 | 188.235 | 184.615 | 181.132 | 177.778 | 174.545 | 171.429 | 168.421 | 165.517 | 162.712 | 160 | 157.377 | 154.839 | 152.381 | 150 | 147.692 | 145.455 | 143.284 | 141.176 | 139.13 | 137.143 | 135.211 | 133.333 | 131.507 | 129.73 | 128 | 126.316 | 124.675 | 123.077 | 121.519 | 120 | 118.519 | 117.073 | 115.663 | 114.286 | 112.941 | 111.628 | 110.345 | 109.091 | 107.865 | 106.667 | 105.495 | 104.348 | 103.226
      mask Callback t225_QT_adc0_enable: enable_adc_opt(gcb,225,0,'QT');
      mask TypeOptions t225_QT_adc0_digital_output: Real | I/Q
      mask Callback t225_QT_adc0_digital_output:
      | validate_digital_data(gcb,225,0,'QT');
      | update_axis_clk(gcb,225);
      mask TypeOptions t225_QT_adc0_dec_mode: 1x | 2x | 3x | 4x | 5x | 6x | 8x | 10x | 12x | 16x | 20x | 24x | 40x
      mask Callback t225_QT_adc0_dec_mode:
      | % if I/Q output mode, need to copy interp factor before updating axis clk
      | % note only the even slice for the tile makes this check
      | if chk_param(gcb, 't225_QT_adc0_mixer_mode', 'I/Q -> I/Q')
      |   dec_mode = get_param(gcb, 't225_QT_adc0_dec_mode');
      |   set_param(gcb, 't225_QT_adc1_dec_mode', dec_mode);
      | end
      | update_axis_clk(gcb,225);
      mask TypeOptions t225_QT_adc0_sample_per_cycle: 4 | 5 | 6 | 7 | 8 | 9 | 10 | 11 | 12
      mask Callback t225_QT_adc0_sample_per_cycle:
      | % if I/Q output mode, need to copy samples per clk before updating axis clk
      | % note only the even slice for the tile makes this check
      | if chk_param(gcb, 't225_QT_adc0_mixer_mode', 'I/Q -> I/Q')
      |   spc = get_param(gcb, 't225_QT_adc0_sample_per_cycle');
      |   set_param(gcb, 't225_QT_adc1_sample_per_cycle', spc);
      | end
      | update_axis_clk_label(gcb,225);
      mask TypeOptions t225_QT_adc0_mixer_type: Bypassed
      mask Callback t225_QT_adc0_mixer_type: mixertype_callback(gcb,225,0,'QT');
      mask TypeOptions t225_QT_adc0_mixer_mode: Real -> Real
      mask Callback t225_QT_adc0_mixer_mode: mixer_callback(gcb,225,0,'QT');
      mask TypeOptions t225_QT_adc0_coarse_freq: 0
      mask TypeOptions t225_QT_adc0_nyquist_zone: Zone 1 | Zone 2
      mask TypeOptions t225_QT_adc0_cal_mode: Mode 1 | Mode 2
      mask Callback t225_QT_adc1_enable: enable_adc_opt(gcb,225,1,'QT');
      mask TypeOptions t225_QT_adc1_digital_output: Real | I/Q
      mask Callback t225_QT_adc1_digital_output:
      | validate_digital_data(gcb,225,1,'QT');
      | update_axis_clk(gcb,225);
      mask TypeOptions t225_QT_adc1_dec_mode: 1x | 2x | 3x | 4x | 5x | 6x | 8x | 10x | 12x | 16x | 20x | 24x | 40x
      mask Callback t225_QT_adc1_dec_mode: update_axis_clk(gcb,225);
      mask TypeOptions t225_QT_adc1_sample_per_cycle: 4 | 5 | 6 | 7 | 8 | 9 | 10 | 11 | 12
      mask Callback t225_QT_adc1_sample_per_cycle: update_axis_clk_label(gcb,225);
      mask TypeOptions t225_QT_adc1_mixer_type: Bypassed
      mask Callback t225_QT_adc1_mixer_type: mixertype_callback(gcb,225,1,'QT');
      mask TypeOptions t225_QT_adc1_mixer_mode: Real -> Real
      mask Callback t225_QT_adc1_mixer_mode: mixer_callback(gcb,225,1,'QT')
      mask TypeOptions t225_QT_adc1_coarse_freq: 0
      mask TypeOptions t225_QT_adc1_nyquist_zone: Zone 1 | Zone 2
      mask TypeOptions t225_QT_adc1_cal_mode: Mode 1 | Mode 2
      mask Callback t225_QT_adc2_enable: enable_adc_opt(gcb,225,2,'QT');
      mask TypeOptions t225_QT_adc2_digital_output: Real | I/Q
      mask Callback t225_QT_adc2_digital_output:
      | validate_digital_data(gcb,225,2,'QT');
      | update_axis_clk(gcb,225);
      mask TypeOptions t225_QT_adc2_dec_mode: 1x | 2x | 3x | 4x | 5x | 6x | 8x | 10x | 12x | 16x | 20x | 24x | 40x
      mask Callback t225_QT_adc2_dec_mode:
      | % if I/Q output mode, need to copy interp factor before updating axis clk
      | % note only the even slice for the tile makes this check
      | if chk_param(gcb, 't225_QT_adc2_mixer_mode', 'I/Q -> I/Q')
      |   dec_mode = get_param(gcb, 't225_QT_adc2_dec_mode');
      |   set_param(gcb, 't225_QT_adc3_dec_mode', dec_mode);
      | end
      | update_axis_clk(gcb,225);
      mask TypeOptions t225_QT_adc2_sample_per_cycle: 4 | 5 | 6 | 7 | 8 | 9 | 10 | 11 | 12
      mask Callback t225_QT_adc2_sample_per_cycle:
      | % if I/Q output mode, need to copy samples per clk before updating axis clk
      | % note only the even slice for the tile makes this check
      | if chk_param(gcb, 't225_QT_adc2_mixer_mode', 'I/Q -> I/Q')
      |   spc = get_param(gcb, 't225_QT_adc2_sample_per_cycle');
      |   set_param(gcb, 't225_QT_adc3_sample_per_cycle', spc);
      | end
      | update_axis_clk_label(gcb,225);
      mask TypeOptions t225_QT_adc2_mixer_type: Bypassed
      mask Callback t225_QT_adc2_mixer_type: mixertype_callback(gcb,225,2,'QT');
      mask TypeOptions t225_QT_adc2_mixer_mode: Real -> Real
      mask Callback t225_QT_adc2_mixer_mode: mixer_callback(gcb,225,2,'QT')
      mask TypeOptions t225_QT_adc2_coarse_freq: 0
      mask TypeOptions t225_QT_adc2_nyquist_zone: Zone 1 | Zone 2
      mask TypeOptions t225_QT_adc2_cal_mode: Mode 1 | Mode 2
      mask Callback t225_QT_adc3_enable: enable_adc_opt(gcb,225,3,'QT');
      mask TypeOptions t225_QT_adc3_digital_output: Real | I/Q
      mask Callback t225_QT_adc3_digital_output:
      | validate_digital_data(gcb,225,3,'QT');
      | update_axis_clk(gcb,225);
      mask TypeOptions t225_QT_adc3_dec_mode: 1x | 2x | 3x | 4x | 5x | 6x | 8x | 10x | 12x | 16x | 20x | 24x | 40x
      mask Callback t225_QT_adc3_dec_mode: update_axis_clk(gcb,225);
      mask TypeOptions t225_QT_adc3_sample_per_cycle: 4 | 5 | 6 | 7 | 8 | 9 | 10 | 11 | 12
      mask Callback t225_QT_adc3_sample_per_cycle: update_axis_clk_label(gcb,225);
      mask TypeOptions t225_QT_adc3_mixer_type: Bypassed
      mask Callback t225_QT_adc3_mixer_type: mixertype_callback(gcb,225,3,'QT');
      mask TypeOptions t225_QT_adc3_mixer_mode: Real -> Real
      mask Callback t225_QT_adc3_mixer_mode: mixer_callback(gcb,225,3,'QT')
      mask TypeOptions t225_QT_adc3_coarse_freq: 0
      mask TypeOptions t225_QT_adc3_nyquist_zone: Zone 1 | Zone 2
      mask TypeOptions t225_QT_adc3_cal_mode: Mode 1 | Mode 2
      mask Callback t225_DT_adc0_enable: enable_adc_opt(gcb,225,0,'DT');
      mask TypeOptions t225_DT_adc0_digital_output: Real | I/Q
      mask Callback t225_DT_adc0_digital_output:
      | validate_digital_data(gcb,225,0,'DT');
      | update_axis_clk(gcb,225);
      mask TypeOptions t225_DT_adc0_dec_mode: 1x | 2x | 3x | 4x | 5x | 6x | 8x | 10x | 12x | 16x | 20x | 24x | 40x
      mask Callback t225_DT_adc0_dec_mode:
      | % if I/Q output mode, need to copy interp factor before updating axis clk
      | % note only the even slice for the tile makes this check
      | if chk_param(gcb, 't225_DT_adc0_mixer_mode', 'I/Q -> I/Q')
      |   dec_mode = get_param(gcb, 't225_DT_adc0_dec_mode');
      |   set_param(gcb, 't225_DT_adc1_dec_mode', dec_mode);
      | end
      | update_axis_clk(gcb,225);
      mask TypeOptions t225_DT_adc0_sample_per_cycle: 5 | 6 | 7 | 8 | 9 | 10 | 11 | 12
      mask Callback t225_DT_adc0_sample_per_cycle:
      | % if I/Q output mode, need to copy samples per clk before updating axis clk
      | % note only the even slice for the tile makes this check
      | if chk_param(gcb, 't225_DT_adc0_mixer_mode', 'I/Q -> I/Q')
      |   spc = get_param(gcb, 't225_DT_adc0_sample_per_cycle');
      |   set_param(gcb, 't225_DT_adc1_sample_per_cycle', spc);
      | end
      | update_axis_clk_label(gcb,225);
      mask TypeOptions t225_DT_adc0_mixer_type: Bypassed
      mask Callback t225_DT_adc0_mixer_type: mixertype_callback(gcb,225,0,'DT');
      mask TypeOptions t225_DT_adc0_mixer_mode: Real -> Real
      mask Callback t225_DT_adc0_mixer_mode: mixer_callback(gcb,225,0,'DT');
      mask TypeOptions t225_DT_adc0_coarse_freq: 0
      mask TypeOptions t225_DT_adc0_nyquist_zone: Zone 1 | Zone 2
      mask TypeOptions t225_DT_adc0_cal_mode: Mode 1 | Mode 2
      mask Callback t225_DT_adc1_enable: enable_adc_opt(gcb,225,1,'DT');
      mask TypeOptions t225_DT_adc1_digital_output: Real | I/Q
      mask Callback t225_DT_adc1_digital_output:
      | validate_digital_data(gcb,225,1,'DT');
      | update_axis_clk(gcb,225);
      mask TypeOptions t225_DT_adc1_dec_mode: 1x | 2x | 3x | 4x | 5x | 6x | 8x | 10x | 12x | 16x | 20x | 24x | 40x
      mask Callback t225_DT_adc1_dec_mode: update_axis_clk(gcb,225);
      mask TypeOptions t225_DT_adc1_sample_per_cycle: 5 | 6 | 7 | 8 | 9 | 10 | 11 | 12
      mask Callback t225_DT_adc1_sample_per_cycle:
      | %update_axis_clk(gcb);
      | update_axis_clk_label(gcb,225);
      mask TypeOptions t225_DT_adc1_mixer_type: Bypassed
      mask Callback t225_DT_adc1_mixer_type: mixertype_callback(gcb,225,1,'DT');
      mask TypeOptions t225_DT_adc1_mixer_mode: Real -> Real
      mask Callback t225_DT_adc1_mixer_mode: mixer_callback(gcb,225,1,'DT');
      mask TypeOptions t225_DT_adc1_coarse_freq: 0
      mask TypeOptions t225_DT_adc1_nyquist_zone: Zone 1 | Zone 2
      mask TypeOptions t225_DT_adc1_cal_mode: Mode 1 | Mode 2
      mask Callback t226_sample_rate: update_rfdc_clocking(gcb,226);
      mask TypeOptions t226_clk_out: 150 | 75 | 37.5 | 18.75
      mask Callback t226_enable_pll:
      | %update_rfdc_clocking(gcb);
      | update_pll(gcb,226);
      mask TypeOptions t226_ref_clk: 738.462 | 685.714 | 640 | 600 | 564.706 | 533.333 | 505.263 | 480 | 457.143 | 436.364 | 417.391 | 400 | 384 | 369.231 | 355.556 | 342.857 | 331.034 | 320 | 309.677 | 300 | 290.909 | 282.353 | 274.286 | 266.667 | 259.459 | 252.632 | 246.154 | 240 | 234.146 | 228.571 | 223.256 | 218.182 | 213.333 | 208.696 | 204.255 | 200 | 195.918 | 192 | 188.235 | 184.615 | 181.132 | 177.778 | 174.545 | 171.429 | 168.421 | 165.517 | 162.712 | 160 | 157.377 | 154.839 | 152.381 | 150 | 147.692 | 145.455 | 143.284 | 141.176 | 139.13 | 137.143 | 135.211 | 133.333 | 131.507 | 129.73 | 128 | 126.316 | 124.675 | 123.077 | 121.519 | 120 | 118.519 | 117.073 | 115.663 | 114.286 | 112.941 | 111.628 | 110.345 | 109.091 | 107.865 | 106.667 | 105.495 | 104.348 | 103.226
      mask Callback t226_QT_adc0_enable: enable_adc_opt(gcb,226,0,'QT');
      mask TypeOptions t226_QT_adc0_digital_output: Real | I/Q
      mask Callback t226_QT_adc0_digital_output:
      | validate_digital_data(gcb,226,0,'QT');
      | update_axis_clk(gcb,226);
      mask TypeOptions t226_QT_adc0_dec_mode: 1x | 2x | 3x | 4x | 5x | 6x | 8x | 10x | 12x | 16x | 20x | 24x | 40x
      mask Callback t226_QT_adc0_dec_mode:
      | % if I/Q output mode, need to copy interp factor before updating axis clk
      | % note only the even slice for the tile makes this check
      | if chk_param(gcb, 't226_QT_adc0_mixer_mode', 'I/Q -> I/Q')
      |   dec_mode = get_param(gcb, 't226_QT_adc0_dec_mode');
      |   set_param(gcb, 't226_QT_adc1_dec_mode', dec_mode);
      | end
      | update_axis_clk(gcb,226);
      mask TypeOptions t226_QT_adc0_sample_per_cycle: 4 | 5 | 6 | 7 | 8 | 9 | 10 | 11 | 12
      mask Callback t226_QT_adc0_sample_per_cycle:
      | % if I/Q output mode, need to copy samples per clk before updating axis clk
      | % note only the even slice for the tile makes this check
      | if chk_param(gcb, 't226_QT_adc0_mixer_mode', 'I/Q -> I/Q')
      |   spc = get_param(gcb, 't226_QT_adc0_sample_per_cycle');
      |   set_param(gcb, 't226_QT_adc1_sample_per_cycle', spc);
      | end
      | update_axis_clk_label(gcb,226);
      mask TypeOptions t226_QT_adc0_mixer_type: Bypassed
      mask Callback t226_QT_adc0_mixer_type: mixertype_callback(gcb,226,0,'QT');
      mask TypeOptions t226_QT_adc0_mixer_mode: Real -> Real
      mask Callback t226_QT_adc0_mixer_mode: mixer_callback(gcb,226,0,'QT');
      mask TypeOptions t226_QT_adc0_coarse_freq: 0
      mask TypeOptions t226_QT_adc0_nyquist_zone: Zone 1 | Zone 2
      mask TypeOptions t226_QT_adc0_cal_mode: Mode 1 | Mode 2
      mask Callback t226_QT_adc1_enable: enable_adc_opt(gcb,226,1,'QT');
      mask TypeOptions t226_QT_adc1_digital_output: Real | I/Q
      mask Callback t226_QT_adc1_digital_output:
      | validate_digital_data(gcb,226,1,'QT');
      | update_axis_clk(gcb,226);
      mask TypeOptions t226_QT_adc1_dec_mode: 1x | 2x | 3x | 4x | 5x | 6x | 8x | 10x | 12x | 16x | 20x | 24x | 40x
      mask Callback t226_QT_adc1_dec_mode: update_axis_clk(gcb,226);
      mask TypeOptions t226_QT_adc1_sample_per_cycle: 4 | 5 | 6 | 7 | 8 | 9 | 10 | 11 | 12
      mask Callback t226_QT_adc1_sample_per_cycle: update_axis_clk_label(gcb,226);
      mask TypeOptions t226_QT_adc1_mixer_type: Bypassed
      mask Callback t226_QT_adc1_mixer_type: mixertype_callback(gcb,226,1,'QT');
      mask TypeOptions t226_QT_adc1_mixer_mode: Real -> Real
      mask Callback t226_QT_adc1_mixer_mode: mixer_callback(gcb,226,1,'QT')
      mask TypeOptions t226_QT_adc1_coarse_freq: 0
      mask TypeOptions t226_QT_adc1_nyquist_zone: Zone 1 | Zone 2
      mask TypeOptions t226_QT_adc1_cal_mode: Mode 1 | Mode 2
      mask Callback t226_QT_adc2_enable: enable_adc_opt(gcb,226,2,'QT');
      mask TypeOptions t226_QT_adc2_digital_output: Real | I/Q
      mask Callback t226_QT_adc2_digital_output:
      | validate_digital_data(gcb,226,2,'QT');
      | update_axis_clk(gcb,226);
      mask TypeOptions t226_QT_adc2_dec_mode: 1x | 2x | 3x | 4x | 5x | 6x | 8x | 10x | 12x | 16x | 20x | 24x | 40x
      mask Callback t226_QT_adc2_dec_mode:
      | % if I/Q output mode, need to copy interp factor before updating axis clk
      | % note only the even slice for the tile makes this check
      | if chk_param(gcb, 't226_QT_adc2_mixer_mode', 'I/Q -> I/Q')
      |   dec_mode = get_param(gcb, 't226_QT_adc2_dec_mode');
      |   set_param(gcb, 't226_QT_adc3_dec_mode', dec_mode);
      | end
      | update_axis_clk(gcb,226);
      mask TypeOptions t226_QT_adc2_sample_per_cycle: 4 | 5 | 6 | 7 | 8 | 9 | 10 | 11 | 12
      mask Callback t226_QT_adc2_sample_per_cycle:
      | % if I/Q output mode, need to copy samples per clk before updating axis clk
      | % note only the even slice for the tile makes this check
      | if chk_param(gcb, 't226_QT_adc2_mixer_mode', 'I/Q -> I/Q')
      |   spc = get_param(gcb, 't226_QT_adc2_sample_per_cycle');
      |   set_param(gcb, 't226_QT_adc3_sample_per_cycle', spc);
      | end
      | update_axis_clk_label(gcb,226);
      mask TypeOptions t226_QT_adc2_mixer_type: Bypassed
      mask Callback t226_QT_adc2_mixer_type: mixertype_callback(gcb,226,2,'QT');
      mask TypeOptions t226_QT_adc2_mixer_mode: Real -> Real
      mask Callback t226_QT_adc2_mixer_mode: mixer_callback(gcb,226,2,'QT')
      mask TypeOptions t226_QT_adc2_coarse_freq: 0
      mask TypeOptions t226_QT_adc2_nyquist_zone: Zone 1 | Zone 2
      mask TypeOptions t226_QT_adc2_cal_mode: Mode 1 | Mode 2
      mask Callback t226_QT_adc3_enable: enable_adc_opt(gcb,226,3,'QT');
      mask TypeOptions t226_QT_adc3_digital_output: Real | I/Q
      mask Callback t226_QT_adc3_digital_output:
      | validate_digital_data(gcb,226,3,'QT');
      | update_axis_clk(gcb,226);
      mask TypeOptions t226_QT_adc3_dec_mode: 1x | 2x | 3x | 4x | 5x | 6x | 8x | 10x | 12x | 16x | 20x | 24x | 40x
      mask Callback t226_QT_adc3_dec_mode: update_axis_clk(gcb,226);
      mask TypeOptions t226_QT_adc3_sample_per_cycle: 4 | 5 | 6 | 7 | 8 | 9 | 10 | 11 | 12
      mask Callback t226_QT_adc3_sample_per_cycle: update_axis_clk_label(gcb,226);
      mask TypeOptions t226_QT_adc3_mixer_type: Bypassed
      mask Callback t226_QT_adc3_mixer_type: mixertype_callback(gcb,226,3,'QT');
      mask TypeOptions t226_QT_adc3_mixer_mode: Real -> Real
      mask Callback t226_QT_adc3_mixer_mode: mixer_callback(gcb,226,3,'QT')
      mask TypeOptions t226_QT_adc3_coarse_freq: 0
      mask TypeOptions t226_QT_adc3_nyquist_zone: Zone 1 | Zone 2
      mask TypeOptions t226_QT_adc3_cal_mode: Mode 1 | Mode 2
      mask Callback t226_DT_adc0_enable: enable_adc_opt(gcb,226,0,'DT');
      mask TypeOptions t226_DT_adc0_digital_output: Real | I/Q
      mask Callback t226_DT_adc0_digital_output:
      | validate_digital_data(gcb,226,0,'DT');
      | update_axis_clk(gcb,226);
      mask TypeOptions t226_DT_adc0_dec_mode: 1x | 2x | 3x | 4x | 5x | 6x | 8x | 10x | 12x | 16x | 20x | 24x | 40x
      mask Callback t226_DT_adc0_dec_mode:
      | % if I/Q output mode, need to copy interp factor before updating axis clk
      | % note only the even slice for the tile makes this check
      | if chk_param(gcb, 't226_DT_adc0_mixer_mode', 'I/Q -> I/Q')
      |   dec_mode = get_param(gcb, 't226_DT_adc0_dec_mode');
      |   set_param(gcb, 't226_DT_adc1_dec_mode', dec_mode);
      | end
      | update_axis_clk(gcb,226);
      mask TypeOptions t226_DT_adc0_sample_per_cycle: 5 | 6 | 7 | 8 | 9 | 10 | 11 | 12
      mask Callback t226_DT_adc0_sample_per_cycle:
      | % if I/Q output mode, need to copy samples per clk before updating axis clk
      | % note only the even slice for the tile makes this check
      | if chk_param(gcb, 't226_DT_adc0_mixer_mode', 'I/Q -> I/Q')
      |   spc = get_param(gcb, 't226_DT_adc0_sample_per_cycle');
      |   set_param(gcb, 't226_DT_adc1_sample_per_cycle', spc);
      | end
      | update_axis_clk_label(gcb,226);
      mask TypeOptions t226_DT_adc0_mixer_type: Bypassed
      mask Callback t226_DT_adc0_mixer_type: mixertype_callback(gcb,226,0,'DT');
      mask TypeOptions t226_DT_adc0_mixer_mode: Real -> Real
      mask Callback t226_DT_adc0_mixer_mode: mixer_callback(gcb,226,0,'DT');
      mask TypeOptions t226_DT_adc0_coarse_freq: 0
      mask TypeOptions t226_DT_adc0_nyquist_zone: Zone 1 | Zone 2
      mask TypeOptions t226_DT_adc0_cal_mode: Mode 1 | Mode 2
      mask Callback t226_DT_adc1_enable: enable_adc_opt(gcb,226,1,'DT');
      mask TypeOptions t226_DT_adc1_digital_output: Real | I/Q
      mask Callback t226_DT_adc1_digital_output:
      | validate_digital_data(gcb,226,1,'DT');
      | update_axis_clk(gcb,226);
      mask TypeOptions t226_DT_adc1_dec_mode: 1x | 2x | 3x | 4x | 5x | 6x | 8x | 10x | 12x | 16x | 20x | 24x | 40x
      mask Callback t226_DT_adc1_dec_mode: update_axis_clk(gcb,226);
      mask TypeOptions t226_DT_adc1_sample_per_cycle: 5 | 6 | 7 | 8 | 9 | 10 | 11 | 12
      mask Callback t226_DT_adc1_sample_per_cycle:
      | %update_axis_clk(gcb);
      | update_axis_clk_label(gcb,226);
      mask TypeOptions t226_DT_adc1_mixer_type: Bypassed
      mask Callback t226_DT_adc1_mixer_type: mixertype_callback(gcb,226,1,'DT');
      mask TypeOptions t226_DT_adc1_mixer_mode: Real -> Real
      mask Callback t226_DT_adc1_mixer_mode: mixer_callback(gcb,226,1,'DT');
      mask TypeOptions t226_DT_adc1_coarse_freq: 0
      mask TypeOptions t226_DT_adc1_nyquist_zone: Zone 1 | Zone 2
      mask TypeOptions t226_DT_adc1_cal_mode: Mode 1 | Mode 2
      mask Callback t227_sample_rate: update_rfdc_clocking(gcb,227);
      mask TypeOptions t227_clk_out: 150 | 75 | 37.5 | 18.75
      mask Callback t227_enable_pll:
      | %update_rfdc_clocking(gcb);
      | update_pll(gcb,227);
      mask TypeOptions t227_ref_clk: 738.462 | 685.714 | 640 | 600 | 564.706 | 533.333 | 505.263 | 480 | 457.143 | 436.364 | 417.391 | 400 | 384 | 369.231 | 355.556 | 342.857 | 331.034 | 320 | 309.677 | 300 | 290.909 | 282.353 | 274.286 | 266.667 | 259.459 | 252.632 | 246.154 | 240 | 234.146 | 228.571 | 223.256 | 218.182 | 213.333 | 208.696 | 204.255 | 200 | 195.918 | 192 | 188.235 | 184.615 | 181.132 | 177.778 | 174.545 | 171.429 | 168.421 | 165.517 | 162.712 | 160 | 157.377 | 154.839 | 152.381 | 150 | 147.692 | 145.455 | 143.284 | 141.176 | 139.13 | 137.143 | 135.211 | 133.333 | 131.507 | 129.73 | 128 | 126.316 | 124.675 | 123.077 | 121.519 | 120 | 118.519 | 117.073 | 115.663 | 114.286 | 112.941 | 111.628 | 110.345 | 109.091 | 107.865 | 106.667 | 105.495 | 104.348 | 103.226
      mask Callback t227_QT_adc0_enable: enable_adc_opt(gcb,227,0,'QT');
      mask TypeOptions t227_QT_adc0_digital_output: Real | I/Q
      mask Callback t227_QT_adc0_digital_output:
      | validate_digital_data(gcb,227,0,'QT');
      | update_axis_clk(gcb,227);
      mask TypeOptions t227_QT_adc0_dec_mode: 1x | 2x | 3x | 4x | 5x | 6x | 8x | 10x | 12x | 16x | 20x | 24x | 40x
      mask Callback t227_QT_adc0_dec_mode:
      | % if I/Q output mode, need to copy interp factor before updating axis clk
      | % note only the even slice for the tile makes this check
      | if chk_param(gcb, 't227_QT_adc0_mixer_mode', 'I/Q -> I/Q')
      |   dec_mode = get_param(gcb, 't227_QT_adc0_dec_mode');
      |   set_param(gcb, 't227_QT_adc1_dec_mode', dec_mode);
      | end
      | update_axis_clk(gcb,227);
      mask TypeOptions t227_QT_adc0_sample_per_cycle: 4 | 5 | 6 | 7 | 8 | 9 | 10 | 11 | 12
      mask Callback t227_QT_adc0_sample_per_cycle:
      | % if I/Q output mode, need to copy samples per clk before updating axis clk
      | % note only the even slice for the tile makes this check
      | if chk_param(gcb, 't227_QT_adc0_mixer_mode', 'I/Q -> I/Q')
      |   spc = get_param(gcb, 't227_QT_adc0_sample_per_cycle');
      |   set_param(gcb, 't227_QT_adc1_sample_per_cycle', spc);
      | end
      | update_axis_clk_label(gcb,227);
      mask TypeOptions t227_QT_adc0_mixer_type: Bypassed
      mask Callback t227_QT_adc0_mixer_type: mixertype_callback(gcb,227,0,'QT');
      mask TypeOptions t227_QT_adc0_mixer_mode: Real -> Real
      mask Callback t227_QT_adc0_mixer_mode: mixer_callback(gcb,227,0,'QT');
      mask TypeOptions t227_QT_adc0_coarse_freq: 0
      mask TypeOptions t227_QT_adc0_nyquist_zone: Zone 1 | Zone 2
      mask TypeOptions t227_QT_adc0_cal_mode: Mode 1 | Mode 2
      mask Callback t227_QT_adc1_enable: enable_adc_opt(gcb,227,1,'QT');
      mask TypeOptions t227_QT_adc1_digital_output: Real | I/Q
      mask Callback t227_QT_adc1_digital_output:
      | validate_digital_data(gcb,227,1,'QT');
      | update_axis_clk(gcb,227);
      mask TypeOptions t227_QT_adc1_dec_mode: 1x | 2x | 3x | 4x | 5x | 6x | 8x | 10x | 12x | 16x | 20x | 24x | 40x
      mask Callback t227_QT_adc1_dec_mode: update_axis_clk(gcb,227);
      mask TypeOptions t227_QT_adc1_sample_per_cycle: 4 | 5 | 6 | 7 | 8 | 9 | 10 | 11 | 12
      mask Callback t227_QT_adc1_sample_per_cycle: update_axis_clk_label(gcb,227);
      mask TypeOptions t227_QT_adc1_mixer_type: Bypassed
      mask Callback t227_QT_adc1_mixer_type: mixertype_callback(gcb,227,1,'QT');
      mask TypeOptions t227_QT_adc1_mixer_mode: Real -> Real
      mask Callback t227_QT_adc1_mixer_mode: mixer_callback(gcb,227,1,'QT')
      mask TypeOptions t227_QT_adc1_coarse_freq: 0
      mask TypeOptions t227_QT_adc1_nyquist_zone: Zone 1 | Zone 2
      mask TypeOptions t227_QT_adc1_cal_mode: Mode 1 | Mode 2
      mask Callback t227_QT_adc2_enable: enable_adc_opt(gcb,227,2,'QT');
      mask TypeOptions t227_QT_adc2_digital_output: Real | I/Q
      mask Callback t227_QT_adc2_digital_output:
      | validate_digital_data(gcb,227,2,'QT');
      | update_axis_clk(gcb,227);
      mask TypeOptions t227_QT_adc2_dec_mode: 1x | 2x | 3x | 4x | 5x | 6x | 8x | 10x | 12x | 16x | 20x | 24x | 40x
      mask Callback t227_QT_adc2_dec_mode:
      | % if I/Q output mode, need to copy interp factor before updating axis clk
      | % note only the even slice for the tile makes this check
      | if chk_param(gcb, 't227_QT_adc2_mixer_mode', 'I/Q -> I/Q')
      |   dec_mode = get_param(gcb, 't227_QT_adc2_dec_mode');
      |   set_param(gcb, 't227_QT_adc3_dec_mode', dec_mode);
      | end
      | update_axis_clk(gcb,227);
      mask TypeOptions t227_QT_adc2_sample_per_cycle: 4 | 5 | 6 | 7 | 8 | 9 | 10 | 11 | 12
      mask Callback t227_QT_adc2_sample_per_cycle:
      | % if I/Q output mode, need to copy samples per clk before updating axis clk
      | % note only the even slice for the tile makes this check
      | if chk_param(gcb, 't227_QT_adc2_mixer_mode', 'I/Q -> I/Q')
      |   spc = get_param(gcb, 't227_QT_adc2_sample_per_cycle');
      |   set_param(gcb, 't227_QT_adc3_sample_per_cycle', spc);
      | end
      | update_axis_clk_label(gcb,227);
      mask TypeOptions t227_QT_adc2_mixer_type: Bypassed
      mask Callback t227_QT_adc2_mixer_type: mixertype_callback(gcb,227,2,'QT');
      mask TypeOptions t227_QT_adc2_mixer_mode: Real -> Real
      mask Callback t227_QT_adc2_mixer_mode: mixer_callback(gcb,227,2,'QT')
      mask TypeOptions t227_QT_adc2_coarse_freq: 0
      mask TypeOptions t227_QT_adc2_nyquist_zone: Zone 1 | Zone 2
      mask TypeOptions t227_QT_adc2_cal_mode: Mode 1 | Mode 2
      mask Callback t227_QT_adc3_enable: enable_adc_opt(gcb,227,3,'QT');
      mask TypeOptions t227_QT_adc3_digital_output: Real | I/Q
      mask Callback t227_QT_adc3_digital_output:
      | validate_digital_data(gcb,227,3,'QT');
      | update_axis_clk(gcb,227);
      mask TypeOptions t227_QT_adc3_dec_mode: 1x | 2x | 3x | 4x | 5x | 6x | 8x | 10x | 12x | 16x | 20x | 24x | 40x
      mask Callback t227_QT_adc3_dec_mode: update_axis_clk(gcb,227);
      mask TypeOptions t227_QT_adc3_sample_per_cycle: 4 | 5 | 6 | 7 | 8 | 9 | 10 | 11 | 12
      mask Callback t227_QT_adc3_sample_per_cycle: update_axis_clk_label(gcb,227);
      mask TypeOptions t227_QT_adc3_mixer_type: Bypassed
      mask Callback t227_QT_adc3_mixer_type: mixertype_callback(gcb,227,3,'QT');
      mask TypeOptions t227_QT_adc3_mixer_mode: Real -> Real
      mask Callback t227_QT_adc3_mixer_mode: mixer_callback(gcb,227,3,'QT')
      mask TypeOptions t227_QT_adc3_coarse_freq: 0
      mask TypeOptions t227_QT_adc3_nyquist_zone: Zone 1 | Zone 2
      mask TypeOptions t227_QT_adc3_cal_mode: Mode 1 | Mode 2
      mask Callback t227_DT_adc0_enable: enable_adc_opt(gcb,227,0,'DT');
      mask TypeOptions t227_DT_adc0_digital_output: Real | I/Q
      mask Callback t227_DT_adc0_digital_output:
      | validate_digital_data(gcb,227,0,'DT');
      | update_axis_clk(gcb,227);
      mask TypeOptions t227_DT_adc0_dec_mode: 1x | 2x | 3x | 4x | 5x | 6x | 8x | 10x | 12x | 16x | 20x | 24x | 40x
      mask Callback t227_DT_adc0_dec_mode:
      | % if I/Q output mode, need to copy interp factor before updating axis clk
      | % note only the even slice for the tile makes this check
      | if chk_param(gcb, 't227_DT_adc0_mixer_mode', 'I/Q -> I/Q')
      |   dec_mode = get_param(gcb, 't227_DT_adc0_dec_mode');
      |   set_param(gcb, 't227_DT_adc1_dec_mode', dec_mode);
      | end
      | update_axis_clk(gcb,227);
      mask TypeOptions t227_DT_adc0_sample_per_cycle: 5 | 6 | 7 | 8 | 9 | 10 | 11 | 12
      mask Callback t227_DT_adc0_sample_per_cycle:
      | % if I/Q output mode, need to copy samples per clk before updating axis clk
      | % note only the even slice for the tile makes this check
      | if chk_param(gcb, 't227_DT_adc0_mixer_mode', 'I/Q -> I/Q')
      |   spc = get_param(gcb, 't227_DT_adc0_sample_per_cycle');
      |   set_param(gcb, 't227_DT_adc1_sample_per_cycle', spc);
      | end
      | update_axis_clk_label(gcb,227);
      mask TypeOptions t227_DT_adc0_mixer_type: Bypassed
      mask Callback t227_DT_adc0_mixer_type: mixertype_callback(gcb,227,0,'DT');
      mask TypeOptions t227_DT_adc0_mixer_mode: Real -> Real
      mask Callback t227_DT_adc0_mixer_mode: mixer_callback(gcb,227,0,'DT');
      mask TypeOptions t227_DT_adc0_coarse_freq: 0
      mask TypeOptions t227_DT_adc0_nyquist_zone: Zone 1 | Zone 2
      mask TypeOptions t227_DT_adc0_cal_mode: Mode 1 | Mode 2
      mask Callback t227_DT_adc1_enable: enable_adc_opt(gcb,227,1,'DT');
      mask TypeOptions t227_DT_adc1_digital_output: Real | I/Q
      mask Callback t227_DT_adc1_digital_output:
      | validate_digital_data(gcb,227,1,'DT');
      | update_axis_clk(gcb,227);
      mask TypeOptions t227_DT_adc1_dec_mode: 1x | 2x | 3x | 4x | 5x | 6x | 8x | 10x | 12x | 16x | 20x | 24x | 40x
      mask Callback t227_DT_adc1_dec_mode: update_axis_clk(gcb,227);
      mask TypeOptions t227_DT_adc1_sample_per_cycle: 5 | 6 | 7 | 8 | 9 | 10 | 11 | 12
      mask Callback t227_DT_adc1_sample_per_cycle:
      | %update_axis_clk(gcb);
      | update_axis_clk_label(gcb,227);
      mask TypeOptions t227_DT_adc1_mixer_type: Bypassed
      mask Callback t227_DT_adc1_mixer_type: mixertype_callback(gcb,227,1,'DT');
      mask TypeOptions t227_DT_adc1_mixer_mode: Real -> Real
      mask Callback t227_DT_adc1_mixer_mode: mixer_callback(gcb,227,1,'DT');
      mask TypeOptions t227_DT_adc1_coarse_freq: 0
      mask TypeOptions t227_DT_adc1_nyquist_zone: Zone 1 | Zone 2
      mask TypeOptions t227_DT_adc1_cal_mode: Mode 1 | Mode 2
      mask Callback t228_sample_rate: update_rfdc_clocking(gcb,228);
      mask TypeOptions t228_clk_out: 125 | 62.5 | 31.25 | 15.625
      mask Callback t228_enable_pll:
      | %update_rfdc_clocking(gcb);
      | update_pll(gcb,228);
      mask TypeOptions t228_ref_clk: 2000
      mask Callback t228_QT_dac0_enable: enable_dac_opt(gcb,228,0,'QT');
      mask TypeOptions t228_QT_dac0_analog_output: Real | I/Q
      mask Callback t228_QT_dac0_analog_output:
      | validate_analog_data(gcb,228,0,'QT');
      | update_axis_clk(gcb,228);
      mask TypeOptions t228_QT_dac0_inter_mode: 1x | 2x | 3x | 4x | 5x | 6x | 8x | 10x | 12x | 16x | 20x | 24x | 40x
      mask Callback t228_QT_dac0_inter_mode:
      | % if I/Q output mode, need to copy interp factor before updating axis clk
      | % note only the even slice for the tile makes this check
      | if chk_param(gcb, 't228_QT_dac0_analog_output', 'I/Q')
      |   inter_mode = get_param(gcb, 't228_QT_dac0_inter_mode');
      |   set_param(gcb, 't228_QT_dac1_inter_mode', inter_mode);
      | end
      | 
      | update_axis_clk(gcb,228);
      mask TypeOptions t228_QT_dac0_sample_per_cycle: 4 | 5 | 6 | 7 | 8 | 9 | 10 | 11 | 12 | 13 | 14 | 15 | 16
      mask Callback t228_QT_dac0_sample_per_cycle:
      | % if I/Q output mode, need to copy samples per clk before updating axis clk
      | if chk_param(gcb, 't228_QT_dac0_analog_output', 'I/Q')
      |   spc = get_param(gcb, 't228_QT_dac0_sample_per_cycle');
      |   set_param(gcb, 't228_QT_dac1_sample_per_cycle', spc);
      | end
      | 
      | update_axis_clk_label(gcb,228);
      mask TypeOptions t228_QT_dac0_datapath_mode: DUC 0 to Fs/2 | DUC 0 to Fs/4 | DUC Fs/4 to Fs/2 | No DUC 0 to Fs/2
      mask TypeOptions t228_QT_dac0_mixer_type: Fine | Coarse
      mask Callback t228_QT_dac0_mixer_type: mixertype_callback(gcb,228,0,'QT');
      mask TypeOptions t228_QT_dac0_mixer_mode: Real -> Real | I/Q -> Real
      mask Callback t228_QT_dac0_mixer_mode: mixer_callback(gcb,228,0,'QT');
      mask TypeOptions t228_QT_dac0_coarse_freq: 0
      mask TypeOptions t228_QT_dac0_nyquist_zone: Zone 1 | Zone 2
      mask TypeOptions t228_QT_dac0_decode_mode: SNR Optimized | Linearity Optimized
      mask Callback t228_QT_dac1_enable: enable_dac_opt(gcb,228,1,'QT');
      mask TypeOptions t228_QT_dac1_analog_output: Real | I/Q
      mask Callback t228_QT_dac1_analog_output:
      | validate_analog_data(gcb,228,1,'QT');
      | update_axis_clk(gcb,228);
      mask TypeOptions t228_QT_dac1_inter_mode: 1x | 2x | 3x | 4x | 5x | 6x | 8x | 10x | 12x | 16x | 20x | 24x | 40x
      mask Callback t228_QT_dac1_inter_mode: update_axis_clk(gcb,228);
      mask TypeOptions t228_QT_dac1_sample_per_cycle: 4 | 5 | 6 | 7 | 8 | 9 | 10 | 11 | 12 | 13 | 14 | 15 | 16
      mask Callback t228_QT_dac1_sample_per_cycle: update_axis_clk_label(gcb,228);
      mask TypeOptions t228_QT_dac1_datapath_mode: DUC 0 to Fs/2 | DUC 0 to Fs/4 | DUC Fs/4 to Fs/2 | No DUC 0 to Fs/2
      mask TypeOptions t228_QT_dac1_mixer_type: Fine | Coarse
      mask Callback t228_QT_dac1_mixer_type: mixertype_callback(gcb,228,1,'QT');
      mask TypeOptions t228_QT_dac1_mixer_mode: Real -> Real | I/Q -> Real
      mask Callback t228_QT_dac1_mixer_mode: mixer_callback(gcb,228,1,'QT')
      mask TypeOptions t228_QT_dac1_coarse_freq: 0
      mask TypeOptions t228_QT_dac1_nyquist_zone: Zone 1 | Zone 2
      mask TypeOptions t228_QT_dac1_decode_mode: SNR Optimized | Linearity Optimized
      mask Callback t228_QT_dac2_enable: enable_dac_opt(gcb,228,2,'QT');
      mask TypeOptions t228_QT_dac2_analog_output: Real | I/Q
      mask Callback t228_QT_dac2_analog_output:
      | validate_analog_data(gcb,228,2,'QT');
      | update_axis_clk(gcb,228);
      mask TypeOptions t228_QT_dac2_inter_mode: 1x | 2x | 3x | 4x | 5x | 6x | 8x | 10x | 12x | 16x | 20x | 24x | 40x
      mask Callback t228_QT_dac2_inter_mode:
      | % if I/Q output mode, need to copy interp factor before updating axis clk
      | % note only the even slice for the tile makes this check
      | if chk_param(gcb, 't228_QT_dac2_analog_output', 'I/Q')
      |   inter_mode = get_param(gcb, 't228_QT_dac2_inter_mode');
      |   set_param(gcb, 't228_QT_dac3_inter_mode', inter_mode);
      | end
      | update_axis_clk(gcb,228);
      mask TypeOptions t228_QT_dac2_sample_per_cycle: 4 | 5 | 6 | 7 | 8 | 9 | 10 | 11 | 12 | 13 | 14 | 15 | 16
      mask Callback t228_QT_dac2_sample_per_cycle:
      | % if I/Q output mode, need to copy samples per clk before updating axis clk
      | % note only the even slice for the tile makes this check
      | if chk_param(gcb, 't228_QT_dac2_analog_output', 'I/Q')
      |   spc = get_param(gcb, 't228_QT_dac2_sample_per_cycle');
      |   set_param(gcb, 't228_QT_dac3_sample_per_cycle', spc);
      | end
      | update_axis_clk_label(gcb,228);
      mask TypeOptions t228_QT_dac2_datapath_mode: DUC 0 to Fs/2 | DUC 0 to Fs/4 | DUC Fs/4 to Fs/2 | No DUC 0 to Fs/2
      mask TypeOptions t228_QT_dac2_mixer_type: Fine | Coarse
      mask Callback t228_QT_dac2_mixer_type: mixertype_callback(gcb,228,2,'QT');
      mask TypeOptions t228_QT_dac2_mixer_mode: Real -> Real | I/Q -> Real
      mask Callback t228_QT_dac2_mixer_mode: mixer_callback(gcb,228,2,'QT')
      mask TypeOptions t228_QT_dac2_coarse_freq: 0
      mask TypeOptions t228_QT_dac2_nyquist_zone: Zone 1 | Zone 2
      mask TypeOptions t228_QT_dac2_decode_mode: SNR Optimized | Linearity Optimized
      mask Callback t228_QT_dac3_enable: enable_dac_opt(gcb,228,3,'QT');
      mask TypeOptions t228_QT_dac3_analog_output: Real | I/Q
      mask Callback t228_QT_dac3_analog_output:
      | validate_analog_data(gcb,228,3,'QT');
      | update_axis_clk(gcb,228);
      mask TypeOptions t228_QT_dac3_inter_mode: 1x | 2x | 3x | 4x | 5x | 6x | 8x | 10x | 12x | 16x | 20x | 24x | 40x
      mask Callback t228_QT_dac3_inter_mode: update_axis_clk(gcb,228);
      mask TypeOptions t228_QT_dac3_sample_per_cycle: 4 | 5 | 6 | 7 | 8 | 9 | 10 | 11 | 12 | 13 | 14 | 15 | 16
      mask Callback t228_QT_dac3_sample_per_cycle: update_axis_clk_label(gcb,228);
      mask TypeOptions t228_QT_dac3_datapath_mode: DUC 0 to Fs/2 | DUC 0 to Fs/4 | DUC Fs/4 to Fs/2 | No DUC 0 to Fs/2
      mask TypeOptions t228_QT_dac3_mixer_type: Fine | Coarse
      mask Callback t228_QT_dac3_mixer_type: mixertype_callback(gcb,228,3,'QT');
      mask TypeOptions t228_QT_dac3_mixer_mode: Real -> Real | I/Q -> Real
      mask Callback t228_QT_dac3_mixer_mode: mixer_callback(gcb,228,3,'QT')
      mask TypeOptions t228_QT_dac3_coarse_freq: 0
      mask TypeOptions t228_QT_dac3_nyquist_zone: Zone 1 | Zone 2
      mask TypeOptions t228_QT_dac3_decode_mode: SNR Optimized | Linearity Optimized
      mask Callback t228_DT_dac0_enable: enable_dac_opt(gcb,228,0,'DT');
      mask TypeOptions t228_DT_dac0_analog_output: Real | I/Q
      mask Callback t228_DT_dac0_analog_output:
      | validate_analog_data(gcb,228,0,'DT');
      | update_axis_clk(gcb,228);
      mask TypeOptions t228_DT_dac0_inter_mode: 1x | 2x | 3x | 4x | 5x | 6x | 8x | 10x | 12x | 16x | 20x | 24x | 40x
      mask Callback t228_DT_dac0_inter_mode:
      | % if I/Q output mode, need to copy interp factor before updating axis clk
      | % note only the even slice for the tile makes this check
      | if chk_param(gcb, 't228_DT_dac0_analog_output', 'I/Q')
      |   inter_mode = get_param(gcb, 't228_DT_dac0_inter_mode');
      |   set_param(gcb, 't228_DT_dac1_inter_mode', inter_mode);
      | end
      | 
      | update_axis_clk(gcb,228);
      mask TypeOptions t228_DT_dac0_sample_per_cycle: 4 | 5 | 6 | 7 | 8 | 9 | 10 | 11 | 12 | 13 | 14 | 15 | 16
      mask Callback t228_DT_dac0_sample_per_cycle:
      | % if I/Q output mode, need to copy samples per clk before updating axis clk
      | if chk_param(gcb, 't228_DT_dac0_analog_output', 'I/Q')
      |   spc = get_param(gcb, 't228_DT_dac0_sample_per_cycle');
      |   set_param(gcb, 't228_DT_dac1_sample_per_cycle', spc);
      | end
      | update_axis_clk_label(gcb,228);
      mask TypeOptions t228_DT_dac0_mixer_type: Fine | Coarse
      mask Callback t228_DT_dac0_mixer_type: mixertype_callback(gcb,228,0,'DT');
      mask TypeOptions t228_DT_dac0_mixer_mode: Real -> Real | I/Q -> Real
      mask Callback t228_DT_dac0_mixer_mode: mixer_callback(gcb,228,0,'DT');
      mask TypeOptions t228_DT_dac0_coarse_freq: 0
      mask TypeOptions t228_DT_dac0_nyquist_zone: Zone 1 | Zone 2
      mask TypeOptions t228_DT_dac0_decode_mode: SNR Optimized | Linearity Optimized
      mask Callback t228_DT_dac1_enable: enable_dac_opt(gcb,228,1,'DT');
      mask TypeOptions t228_DT_dac1_analog_output: Real
      mask Callback t228_DT_dac1_analog_output:
      | validate_analog_data(gcb,228,1,'DT');
      | update_axis_clk(gcb,228);
      mask TypeOptions t228_DT_dac1_inter_mode: 1x | 2x | 3x | 4x | 5x | 6x | 8x | 10x | 12x | 16x | 20x | 24x | 40x
      mask Callback t228_DT_dac1_inter_mode: update_axis_clk(gcb,228);
      mask TypeOptions t228_DT_dac1_sample_per_cycle: 4 | 5 | 6 | 7 | 8 | 9 | 10 | 11 | 12 | 13 | 14 | 15 | 16
      mask Callback t228_DT_dac1_sample_per_cycle:
      | %update_axis_clk(gcb);
      | update_axis_clk_label(gcb,228);
      mask TypeOptions t228_DT_dac1_mixer_type: Fine | Coarse
      mask Callback t228_DT_dac1_mixer_type: mixertype_callback(gcb,228,1,'DT');
      mask TypeOptions t228_DT_dac1_mixer_mode: Real -> Real | I/Q -> Real
      mask Callback t228_DT_dac1_mixer_mode: mixer_callback(gcb,228,1,'DT');
      mask TypeOptions t228_DT_dac1_coarse_freq: 0
      mask TypeOptions t228_DT_dac1_nyquist_zone: Zone 1 | Zone 2
      mask TypeOptions t228_DT_dac1_decode_mode: SNR Optimized | Linearity Optimized
      mask Callback t229_sample_rate: update_rfdc_clocking(gcb,229);
      mask TypeOptions t229_clk_out: 125 | 62.5 | 31.25 | 15.625
      mask Callback t229_enable_pll:
      | %update_rfdc_clocking(gcb);
      | update_pll(gcb,229);
      mask TypeOptions t229_ref_clk: 2000
      mask Callback t229_QT_dac0_enable: enable_dac_opt(gcb,229,0,'QT');
      mask TypeOptions t229_QT_dac0_analog_output: Real | I/Q
      mask Callback t229_QT_dac0_analog_output:
      | validate_analog_data(gcb,229,0,'QT');
      | update_axis_clk(gcb,229);
      mask TypeOptions t229_QT_dac0_inter_mode: 1x | 2x | 3x | 4x | 5x | 6x | 8x | 10x | 12x | 16x | 20x | 24x | 40x
      mask Callback t229_QT_dac0_inter_mode:
      | % if I/Q output mode, need to copy interp factor before updating axis clk
      | % note only the even slice for the tile makes this check
      | if chk_param(gcb, 't229_QT_dac0_analog_output', 'I/Q')
      |   inter_mode = get_param(gcb, 't229_QT_dac0_inter_mode');
      |   set_param(gcb, 't229_QT_dac1_inter_mode', inter_mode);
      | end
      | update_axis_clk(gcb,229);
      mask TypeOptions t229_QT_dac0_sample_per_cycle: 4 | 5 | 6 | 7 | 8 | 9 | 10 | 11 | 12 | 13 | 14 | 15 | 16
      mask Callback t229_QT_dac0_sample_per_cycle:
      | % if I/Q output mode, need to copy samples per clk before updating axis clk
      | % note only the even slice for the tile makes this check
      | if chk_param(gcb, 't229_QT_dac0_analog_output', 'I/Q')
      |   spc = get_param(gcb, 't229_QT_dac0_sample_per_cycle');
      |   set_param(gcb, 't229_QT_dac1_sample_per_cycle', spc);
      | end
      | update_axis_clk_label(gcb,229);
      mask TypeOptions t229_QT_dac0_datapath_mode: DUC 0 to Fs/2 | DUC 0 to Fs/4 | DUC Fs/4 to Fs/2 | No DUC 0 to Fs/2
      mask TypeOptions t229_QT_dac0_mixer_type: Fine | Coarse
      mask Callback t229_QT_dac0_mixer_type: mixertype_callback(gcb,229,0,'QT');
      mask TypeOptions t229_QT_dac0_mixer_mode: Real -> Real | I/Q -> Real
      mask Callback t229_QT_dac0_mixer_mode: mixer_callback(gcb,229,0,'QT');
      mask TypeOptions t229_QT_dac0_coarse_freq: 0
      mask TypeOptions t229_QT_dac0_nyquist_zone: Zone 1 | Zone 2
      mask TypeOptions t229_QT_dac0_decode_mode: SNR Optimized | Linearity Optimized
      mask Callback t229_QT_dac1_enable: enable_dac_opt(gcb,229,1,'QT');
      mask TypeOptions t229_QT_dac1_analog_output: Real
      mask Callback t229_QT_dac1_analog_output:
      | validate_analog_data(gcb,229,1,'QT');
      | update_axis_clk(gcb,229);
      mask TypeOptions t229_QT_dac1_inter_mode: 1x | 2x | 3x | 4x | 5x | 6x | 8x | 10x | 12x | 16x | 20x | 24x | 40x
      mask Callback t229_QT_dac1_inter_mode: update_axis_clk(gcb,229);
      mask TypeOptions t229_QT_dac1_sample_per_cycle: 4 | 5 | 6 | 7 | 8 | 9 | 10 | 11 | 12 | 13 | 14 | 15 | 16
      mask Callback t229_QT_dac1_sample_per_cycle: update_axis_clk_label(gcb,229);
      mask TypeOptions t229_QT_dac1_datapath_mode: DUC 0 to Fs/2 | DUC 0 to Fs/4 | DUC Fs/4 to Fs/2 | No DUC 0 to Fs/2
      mask TypeOptions t229_QT_dac1_mixer_type: Fine | Coarse
      mask Callback t229_QT_dac1_mixer_type: mixertype_callback(gcb,229,1,'QT');
      mask TypeOptions t229_QT_dac1_mixer_mode: Real -> Real | I/Q -> Real
      mask Callback t229_QT_dac1_mixer_mode: mixer_callback(gcb,229,1,'QT')
      mask TypeOptions t229_QT_dac1_coarse_freq: 0
      mask TypeOptions t229_QT_dac1_nyquist_zone: Zone 1 | Zone 2
      mask TypeOptions t229_QT_dac1_decode_mode: SNR Optimized | Linearity Optimized
      mask Callback t229_QT_dac2_enable: enable_dac_opt(gcb,229,2,'QT');
      mask TypeOptions t229_QT_dac2_analog_output: Real | I/Q
      mask Callback t229_QT_dac2_analog_output:
      | validate_analog_data(gcb,229,2,'QT');
      | update_axis_clk(gcb,229);
      mask TypeOptions t229_QT_dac2_inter_mode: 1x | 2x | 3x | 4x | 5x | 6x | 8x | 10x | 12x | 16x | 20x | 24x | 40x
      mask Callback t229_QT_dac2_inter_mode:
      | % if I/Q output mode, need to copy interp factor before updating axis clk
      | % note only the even slice for the tile makes this check
      | if chk_param(gcb, 't229_QT_dac2_analog_output', 'I/Q')
      |   inter_mode = get_param(gcb, 't229_QT_dac2_inter_mode');
      |   set_param(gcb, 't229_QT_dac3_inter_mode', inter_mode);
      | end
      | update_axis_clk(gcb,229);
      mask TypeOptions t229_QT_dac2_sample_per_cycle: 4 | 5 | 6 | 7 | 8 | 9 | 10 | 11 | 12 | 13 | 14 | 15 | 16
      mask Callback t229_QT_dac2_sample_per_cycle:
      | % if I/Q output mode, need to copy samples per clk before updating axis clk
      | % note only the even slice for the tile makes this check
      | if chk_param(gcb, 't229_QT_dac2_analog_output', 'I/Q')
      |   spc = get_param(gcb, 't229_QT_dac2_sample_per_cycle');
      |   set_param(gcb, 't229_QT_dac3_sample_per_cycle', spc);
      | end
      | update_axis_clk_label(gcb,229);
      mask TypeOptions t229_QT_dac2_datapath_mode: DUC 0 to Fs/2 | DUC 0 to Fs/4 | DUC Fs/4 to Fs/2 | No DUC 0 to Fs/2
      mask TypeOptions t229_QT_dac2_mixer_type: Fine | Coarse
      mask Callback t229_QT_dac2_mixer_type: mixertype_callback(gcb,229,2,'QT');
      mask TypeOptions t229_QT_dac2_mixer_mode: Real -> Real | I/Q -> Real
      mask Callback t229_QT_dac2_mixer_mode: mixer_callback(gcb,229,2,'QT')
      mask TypeOptions t229_QT_dac2_coarse_freq: 0
      mask TypeOptions t229_QT_dac2_nyquist_zone: Zone 1 | Zone 2
      mask TypeOptions t229_QT_dac2_decode_mode: SNR Optimized | Linearity Optimized
      mask Callback t229_QT_dac3_enable: enable_dac_opt(gcb,229,3,'QT');
      mask TypeOptions t229_QT_dac3_analog_output: Real | I/Q
      mask Callback t229_QT_dac3_analog_output:
      | validate_analog_data(gcb,229,3,'QT');
      | update_axis_clk(gcb,229);
      mask TypeOptions t229_QT_dac3_inter_mode: 1x | 2x | 3x | 4x | 5x | 6x | 8x | 10x | 12x | 16x | 20x | 24x | 40x
      mask Callback t229_QT_dac3_inter_mode: update_axis_clk(gcb,229);
      mask TypeOptions t229_QT_dac3_sample_per_cycle: 4 | 5 | 6 | 7 | 8 | 9 | 10 | 11 | 12 | 13 | 14 | 15 | 16
      mask Callback t229_QT_dac3_sample_per_cycle: update_axis_clk_label(gcb,229);
      mask TypeOptions t229_QT_dac3_datapath_mode: DUC 0 to Fs/2 | DUC 0 to Fs/4 | DUC Fs/4 to Fs/2 | No DUC 0 to Fs/2
      mask TypeOptions t229_QT_dac3_mixer_type: Fine | Coarse
      mask Callback t229_QT_dac3_mixer_type: mixertype_callback(gcb,229,3,'QT');
      mask TypeOptions t229_QT_dac3_mixer_mode: Real -> Real | I/Q -> Real
      mask Callback t229_QT_dac3_mixer_mode: mixer_callback(gcb,229,3,'QT')
      mask TypeOptions t229_QT_dac3_coarse_freq: 0
      mask TypeOptions t229_QT_dac3_nyquist_zone: Zone 1 | Zone 2
      mask TypeOptions t229_QT_dac3_decode_mode: SNR Optimized | Linearity Optimized
      mask Callback t229_DT_dac0_enable: enable_dac_opt(gcb,229,0,'DT');
      mask TypeOptions t229_DT_dac0_analog_output: Real | I/Q
      mask Callback t229_DT_dac0_analog_output:
      | validate_analog_data(gcb,229,0,'DT');
      | update_axis_clk(gcb,229);
      mask TypeOptions t229_DT_dac0_inter_mode: 1x | 2x | 3x | 4x | 5x | 6x | 8x | 10x | 12x | 16x | 20x | 24x | 40x
      mask Callback t229_DT_dac0_inter_mode:
      | % if I/Q output mode, need to copy interp factor before updating axis clk
      | % note only the even slice for the tile makes this check
      | if chk_param(gcb, 't229_DT_dac0_analog_output', 'I/Q')
      |   inter_mode = get_param(gcb, 't229_DT_dac0_inter_mode');
      |   set_param(gcb, 't229_DT_dac1_inter_mode', inter_mode);
      | end
      | update_axis_clk(gcb,229);
      mask TypeOptions t229_DT_dac0_sample_per_cycle: 4 | 5 | 6 | 7 | 8 | 9 | 10 | 11 | 12 | 13 | 14 | 15 | 16
      mask Callback t229_DT_dac0_sample_per_cycle:
      | % if I/Q output mode, need to copy samples per clk before updating axis clk
      | % note only the even slice for the tile makes this check
      | if chk_param(gcb, 't229_DT_dac0_analog_output', 'I/Q')
      |   spc = get_param(gcb, 't229_DT_dac0_sample_per_cycle');
      |   set_param(gcb, 't229_DT_dac1_sample_per_cycle', spc);
      | end
      | update_axis_clk_label(gcb,229);
      mask TypeOptions t229_DT_dac0_mixer_type: Fine | Coarse
      mask Callback t229_DT_dac0_mixer_type: mixertype_callback(gcb,229,0,'DT');
      mask TypeOptions t229_DT_dac0_mixer_mode: Real -> Real | I/Q -> Real
      mask Callback t229_DT_dac0_mixer_mode: mixer_callback(gcb,229,0,'DT');
      mask TypeOptions t229_DT_dac0_coarse_freq: 0
      mask TypeOptions t229_DT_dac0_nyquist_zone: Zone 1 | Zone 2
      mask TypeOptions t229_DT_dac0_decode_mode: SNR Optimized | Linearity Optimized
      mask Callback t229_DT_dac1_enable: enable_dac_opt(gcb,229,1,'DT');
      mask TypeOptions t229_DT_dac1_analog_output: Real
      mask Callback t229_DT_dac1_analog_output:
      | validate_analog_data(gcb,229,1,'DT');
      | update_axis_clk(gcb,229);
      mask TypeOptions t229_DT_dac1_inter_mode: 1x | 2x | 3x | 4x | 5x | 6x | 8x | 10x | 12x | 16x | 20x | 24x | 40x
      mask Callback t229_DT_dac1_inter_mode: update_axis_clk(gcb,229);
      mask TypeOptions t229_DT_dac1_sample_per_cycle: 4 | 5 | 6 | 7 | 8 | 9 | 10 | 11 | 12 | 13 | 14 | 15 | 16
      mask Callback t229_DT_dac1_sample_per_cycle:
      | %update_axis_clk(gcb);
      | update_axis_clk_label(gcb,229);
      mask TypeOptions t229_DT_dac1_mixer_type: Fine | Coarse
      mask Callback t229_DT_dac1_mixer_type: mixertype_callback(gcb,229,1,'DT');
      mask TypeOptions t229_DT_dac1_mixer_mode: Real -> Real | I/Q -> Real
      mask Callback t229_DT_dac1_mixer_mode: mixer_callback(gcb,229,1,'DT');
      mask TypeOptions t229_DT_dac1_coarse_freq: 0
      mask TypeOptions t229_DT_dac1_nyquist_zone: Zone 1 | Zone 2
      mask TypeOptions t229_DT_dac1_decode_mode: SNR Optimized | Linearity Optimized
      mask Callback t230_sample_rate: update_rfdc_clocking(gcb,230);
      mask TypeOptions t230_clk_out: 125 | 62.5 | 31.25 | 15.625
      mask Callback t230_enable_pll:
      | %update_rfdc_clocking(gcb);
      | update_pll(gcb,230);
      mask TypeOptions t230_ref_clk: 2000
      mask Callback t230_QT_dac0_enable: enable_dac_opt(gcb,230,0,'QT');
      mask TypeOptions t230_QT_dac0_analog_output: Real | I/Q
      mask Callback t230_QT_dac0_analog_output:
      | validate_analog_data(gcb,230,0,'QT');
      | update_axis_clk(gcb,230);
      mask TypeOptions t230_QT_dac0_inter_mode: 1x | 2x | 3x | 4x | 5x | 6x | 8x | 10x | 12x | 16x | 20x | 24x | 40x
      mask Callback t230_QT_dac0_inter_mode:
      | % if I/Q output mode, need to copy interp factor before updating axis clk
      | % note only the even slice for the tile makes this check
      | if chk_param(gcb, 't230_QT_dac0_analog_output', 'I/Q')
      |   inter_mode = get_param(gcb, 't230_QT_dac0_inter_mode');
      |   set_param(gcb, 't230_QT_dac1_inter_mode', inter_mode);
      | end
      | update_axis_clk(gcb,230);
      mask TypeOptions t230_QT_dac0_sample_per_cycle: 4 | 5 | 6 | 7 | 8 | 9 | 10 | 11 | 12 | 13 | 14 | 15 | 16
      mask Callback t230_QT_dac0_sample_per_cycle:
      | % if I/Q output mode, need to copy samples per clk before updating axis clk
      | % note only the even slice for the tile makes this check
      | if chk_param(gcb, 't230_QT_dac0_analog_output', 'I/Q')
      |   spc = get_param(gcb, 't230_QT_dac0_sample_per_cycle');
      |   set_param(gcb, 't230_QT_dac1_sample_per_cycle', spc);
      | end
      | 
      | update_axis_clk_label(gcb,230);
      mask TypeOptions t230_QT_dac0_datapath_mode: DUC 0 to Fs/2 | DUC 0 to Fs/4 | DUC Fs/4 to Fs/2 | No DUC 0 to Fs/2
      mask TypeOptions t230_QT_dac0_mixer_type: Fine | Coarse
      mask Callback t230_QT_dac0_mixer_type: mixertype_callback(gcb,230,0,'QT');
      mask TypeOptions t230_QT_dac0_mixer_mode: Real -> Real | I/Q -> Real
      mask Callback t230_QT_dac0_mixer_mode: mixer_callback(gcb,230,0,'QT');
      mask TypeOptions t230_QT_dac0_coarse_freq: 0
      mask TypeOptions t230_QT_dac0_nyquist_zone: Zone 1 | Zone 2
      mask TypeOptions t230_QT_dac0_decode_mode: SNR Optimized | Linearity Optimized
      mask Callback t230_QT_dac1_enable: enable_dac_opt(gcb,230,1,'QT');
      mask TypeOptions t230_QT_dac1_analog_output: Real | I/Q
      mask Callback t230_QT_dac1_analog_output:
      | validate_analog_data(gcb,230,1,'QT');
      | update_axis_clk(gcb,230);
      mask TypeOptions t230_QT_dac1_inter_mode: 1x | 2x | 3x | 4x | 5x | 6x | 8x | 10x | 12x | 16x | 20x | 24x | 40x
      mask Callback t230_QT_dac1_inter_mode: update_axis_clk(gcb,230);
      mask TypeOptions t230_QT_dac1_sample_per_cycle: 4 | 5 | 6 | 7 | 8 | 9 | 10 | 11 | 12 | 13 | 14 | 15 | 16
      mask Callback t230_QT_dac1_sample_per_cycle: update_axis_clk_label(gcb,230);
      mask TypeOptions t230_QT_dac1_datapath_mode: DUC 0 to Fs/2 | DUC 0 to Fs/4 | DUC Fs/4 to Fs/2 | No DUC 0 to Fs/2
      mask TypeOptions t230_QT_dac1_mixer_type: Fine | Coarse
      mask Callback t230_QT_dac1_mixer_type: mixertype_callback(gcb,230,1,'QT');
      mask TypeOptions t230_QT_dac1_mixer_mode: Real -> Real | I/Q -> Real
      mask Callback t230_QT_dac1_mixer_mode: mixer_callback(gcb,230,1,'QT')
      mask TypeOptions t230_QT_dac1_coarse_freq: 0
      mask TypeOptions t230_QT_dac1_nyquist_zone: Zone 1 | Zone 2
      mask TypeOptions t230_QT_dac1_decode_mode: SNR Optimized | Linearity Optimized
      mask Callback t230_QT_dac2_enable: enable_dac_opt(gcb,230,2,'QT');
      mask TypeOptions t230_QT_dac2_analog_output: Real | I/Q
      mask Callback t230_QT_dac2_analog_output:
      | validate_analog_data(gcb,230,2,'QT');
      | update_axis_clk(gcb,230);
      mask TypeOptions t230_QT_dac2_inter_mode: 1x | 2x | 3x | 4x | 5x | 6x | 8x | 10x | 12x | 16x | 20x | 24x | 40x
      mask Callback t230_QT_dac2_inter_mode:
      | % if I/Q output mode, need to copy interp factor before updating axis clk
      | % note only the even slice for the tile makes this check
      | if chk_param(gcb, 't230_QT_dac2_analog_output', 'I/Q')
      |   inter_mode = get_param(gcb, 't230_QT_dac2_inter_mode');
      |   set_param(gcb, 't230_QT_dac3_inter_mode', inter_mode);
      | end
      | 
      | update_axis_clk(gcb,230);
      mask TypeOptions t230_QT_dac2_sample_per_cycle: 4 | 5 | 6 | 7 | 8 | 9 | 10 | 11 | 12 | 13 | 14 | 15 | 16
      mask Callback t230_QT_dac2_sample_per_cycle:
      | % if I/Q output mode, need to copy samples per clk before updating axis clk
      | % note only the even slice for the tile makes this check
      | if chk_param(gcb, 't230_QT_dac2_analog_output', 'I/Q')
      |   spc = get_param(gcb, 't230_QT_dac2_sample_per_cycle');
      |   set_param(gcb, 't230_QT_dac3_sample_per_cycle', spc);
      | end
      | 
      | update_axis_clk_label(gcb,230)
      mask TypeOptions t230_QT_dac2_datapath_mode: DUC 0 to Fs/2 | DUC 0 to Fs/4 | DUC Fs/4 to Fs/2 | No DUC 0 to Fs/2
      mask TypeOptions t230_QT_dac2_mixer_type: Fine | Coarse
      mask Callback t230_QT_dac2_mixer_type: mixertype_callback(gcb,230,2,'QT');
      mask TypeOptions t230_QT_dac2_mixer_mode: Real -> Real | I/Q -> Real
      mask Callback t230_QT_dac2_mixer_mode: mixer_callback(gcb,230,2,'QT')
      mask TypeOptions t230_QT_dac2_coarse_freq: 0
      mask TypeOptions t230_QT_dac2_nyquist_zone: Zone 1 | Zone 2
      mask TypeOptions t230_QT_dac2_decode_mode: SNR Optimized | Linearity Optimized
      mask Callback t230_QT_dac3_enable: enable_dac_opt(gcb,230,3,'QT');
      mask TypeOptions t230_QT_dac3_analog_output: Real | I/Q
      mask Callback t230_QT_dac3_analog_output:
      | validate_analog_data(gcb,230,3,'QT');
      | update_axis_clk(gcb,230);
      mask TypeOptions t230_QT_dac3_inter_mode: 1x | 2x | 3x | 4x | 5x | 6x | 8x | 10x | 12x | 16x | 20x | 24x | 40x
      mask Callback t230_QT_dac3_inter_mode: update_axis_clk(gcb,230);
      mask TypeOptions t230_QT_dac3_sample_per_cycle: 4 | 5 | 6 | 7 | 8 | 9 | 10 | 11 | 12 | 13 | 14 | 15 | 16
      mask Callback t230_QT_dac3_sample_per_cycle: update_axis_clk_label(gcb,230);
      mask TypeOptions t230_QT_dac3_datapath_mode: DUC 0 to Fs/2 | DUC 0 to Fs/4 | DUC Fs/4 to Fs/2 | No DUC 0 to Fs/2
      mask TypeOptions t230_QT_dac3_mixer_type: Fine | Coarse
      mask Callback t230_QT_dac3_mixer_type: mixertype_callback(gcb,230,3,'QT');
      mask TypeOptions t230_QT_dac3_mixer_mode: Real -> Real | I/Q -> Real
      mask Callback t230_QT_dac3_mixer_mode: mixer_callback(gcb,230,3,'QT')
      mask TypeOptions t230_QT_dac3_coarse_freq: 0
      mask TypeOptions t230_QT_dac3_nyquist_zone: Zone 1 | Zone 2
      mask TypeOptions t230_QT_dac3_decode_mode: SNR Optimized | Linearity Optimized
      mask Callback t230_DT_dac0_enable: enable_dac_opt(gcb,230,0,'DT');
      mask TypeOptions t230_DT_dac0_analog_output: Real | I/Q
      mask Callback t230_DT_dac0_analog_output:
      | validate_analog_data(gcb,230,0,'DT');
      | update_axis_clk(gcb,230);
      mask TypeOptions t230_DT_dac0_inter_mode: 1x | 2x | 3x | 4x | 5x | 6x | 8x | 10x | 12x | 16x | 20x | 24x | 40x
      mask Callback t230_DT_dac0_inter_mode:
      | % if I/Q output mode, need to copy interp factor before updating axis clk
      | % note only the even slice for the tile makes this check
      | if chk_param(gcb, 't230_DT_dac0_analog_output', 'I/Q')
      |   inter_mode = get_param(gcb, 't230_DT_dac0_inter_mode');
      |   set_param(gcb, 't230_DT_dac1_inter_mode', inter_mode);
      | end
      | 
      | update_axis_clk(gcb,230);
      mask TypeOptions t230_DT_dac0_sample_per_cycle: 4 | 5 | 6 | 7 | 8 | 9 | 10 | 11 | 12 | 13 | 14 | 15 | 16
      mask Callback t230_DT_dac0_sample_per_cycle:
      | % if I/Q output mode, need to copy samples per clk before updating axis clk
      | % note only the even slice for the tile makes this check
      | if chk_param(gcb, 't230_DT_dac0_analog_output', 'I/Q')
      |   spc = get_param(gcb, 't230_DT_dac0_sample_per_cycle');
      |   set_param(gcb, 't230_DT_dac1_sample_per_cycle', spc);
      | end
      | update_axis_clk_label(gcb,230);
      mask TypeOptions t230_DT_dac0_mixer_type: Fine | Coarse
      mask Callback t230_DT_dac0_mixer_type: mixertype_callback(gcb,230,0,'DT');
      mask TypeOptions t230_DT_dac0_mixer_mode: Real -> Real | I/Q -> Real
      mask Callback t230_DT_dac0_mixer_mode: mixer_callback(gcb,230,0,'DT');
      mask TypeOptions t230_DT_dac0_coarse_freq: 0
      mask TypeOptions t230_DT_dac0_nyquist_zone: Zone 1 | Zone 2
      mask TypeOptions t230_DT_dac0_decode_mode: SNR Optimized | Linearity Optimized
      mask Callback t230_DT_dac1_enable: enable_dac_opt(gcb,230,1,'DT');
      mask TypeOptions t230_DT_dac1_analog_output: Real
      mask Callback t230_DT_dac1_analog_output:
      | validate_analog_data(gcb,230,1,'DT');
      | update_axis_clk(gcb,229);
      mask TypeOptions t230_DT_dac1_inter_mode: 1x | 2x | 3x | 4x | 5x | 6x | 8x | 10x | 12x | 16x | 20x | 24x | 40x
      mask Callback t230_DT_dac1_inter_mode: update_axis_clk(gcb,230);
      mask TypeOptions t230_DT_dac1_sample_per_cycle: 4 | 5 | 6 | 7 | 8 | 9 | 10 | 11 | 12 | 13 | 14 | 15 | 16
      mask Callback t230_DT_dac1_sample_per_cycle:
      | %update_axis_clk(gcb);
      | update_axis_clk_label(gcb,230);
      mask TypeOptions t230_DT_dac1_mixer_type: Fine | Coarse
      mask Callback t230_DT_dac1_mixer_type: mixertype_callback(gcb,230,1,'DT');
      mask TypeOptions t230_DT_dac1_mixer_mode: Real -> Real | I/Q -> Real
      mask Callback t230_DT_dac1_mixer_mode: mixer_callback(gcb,230,1,'DT');
      mask TypeOptions t230_DT_dac1_coarse_freq: 0
      mask TypeOptions t230_DT_dac1_nyquist_zone: Zone 1 | Zone 2
      mask TypeOptions t230_DT_dac1_decode_mode: SNR Optimized | Linearity Optimized
      mask Callback t231_sample_rate: update_rfdc_clocking(gcb,231);
      mask TypeOptions t231_clk_out: 125 | 62.5 | 31.25 | 15.625
      mask Callback t231_enable_pll:
      | %update_rfdc_clocking(gcb);
      | update_pll(gcb,231);
      mask TypeOptions t231_ref_clk: 2000
      mask Callback t231_QT_dac0_enable: enable_dac_opt(gcb,231,0,'QT');
      mask TypeOptions t231_QT_dac0_analog_output: Real | I/Q
      mask Callback t231_QT_dac0_analog_output:
      | validate_analog_data(gcb,231,0,'QT');
      | update_axis_clk(gcb,231);
      mask TypeOptions t231_QT_dac0_inter_mode: 1x | 2x | 3x | 4x | 5x | 6x | 8x | 10x | 12x | 16x | 20x | 24x | 40x
      mask Callback t231_QT_dac0_inter_mode:
      | % if I/Q output mode, need to copy interp factor before updating axis clk
      | % note only the even slice for the tile makes this check
      | if chk_param(gcb, 't231_QT_dac0_analog_output', 'I/Q')
      |   inter_mode = get_param(gcb, 't231_QT_dac0_inter_mode');
      |   set_param(gcb, 't231_QT_dac1_inter_mode', inter_mode);
      | end
      | update_axis_clk(gcb,231);
      mask TypeOptions t231_QT_dac0_sample_per_cycle: 4 | 5 | 6 | 7 | 8 | 9 | 10 | 11 | 12 | 13 | 14 | 15 | 16
      mask Callback t231_QT_dac0_sample_per_cycle:
      | % if I/Q output mode, need to copy samples per clk before updating axis clk
      | % note only the even slice for the tile makes this check
      | if chk_param(gcb, 't231_QT_dac0_analog_output', 'I/Q')
      |   spc = get_param(gcb, 't231_QT_dac0_sample_per_cycle');
      |   set_param(gcb, 't231_QT_dac1_sample_per_cycle', spc);
      | end
      | update_axis_clk_label(gcb,231);
      mask TypeOptions t231_QT_dac0_datapath_mode: DUC 0 to Fs/2 | DUC 0 to Fs/4 | DUC Fs/4 to Fs/2 | No DUC 0 to Fs/2
      mask TypeOptions t231_QT_dac0_mixer_type: Fine | Coarse
      mask Callback t231_QT_dac0_mixer_type: mixertype_callback(gcb,231,0,'QT');
      mask TypeOptions t231_QT_dac0_mixer_mode: Real -> Real | I/Q -> Real
      mask Callback t231_QT_dac0_mixer_mode: mixer_callback(gcb,231,0,'QT');
      mask TypeOptions t231_QT_dac0_coarse_freq: 0
      mask TypeOptions t231_QT_dac0_nyquist_zone: Zone 1 | Zone 2
      mask TypeOptions t231_QT_dac0_decode_mode: SNR Optimized | Linearity Optimized
      mask Callback t231_QT_dac1_enable: enable_dac_opt(gcb,231,1,'QT');
      mask TypeOptions t231_QT_dac1_analog_output: Real | I/Q
      mask Callback t231_QT_dac1_analog_output:
      | validate_analog_data(gcb,231,1,'QT');
      | update_axis_clk(gcb,231);
      mask TypeOptions t231_QT_dac1_inter_mode: 1x | 2x | 3x | 4x | 5x | 6x | 8x | 10x | 12x | 16x | 20x | 24x | 40x
      mask Callback t231_QT_dac1_inter_mode: update_axis_clk(gcb,231);
      mask TypeOptions t231_QT_dac1_sample_per_cycle: 4 | 5 | 6 | 7 | 8 | 9 | 10 | 11 | 12 | 13 | 14 | 15 | 16
      mask Callback t231_QT_dac1_sample_per_cycle: update_axis_clk_label(gcb,231);
      mask TypeOptions t231_QT_dac1_datapath_mode: DUC 0 to Fs/2 | DUC 0 to Fs/4 | DUC Fs/4 to Fs/2 | No DUC 0 to Fs/2
      mask TypeOptions t231_QT_dac1_mixer_type: Fine | Coarse
      mask Callback t231_QT_dac1_mixer_type: mixertype_callback(gcb,231,1,'QT');
      mask TypeOptions t231_QT_dac1_mixer_mode: Real -> Real | I/Q -> Real
      mask Callback t231_QT_dac1_mixer_mode: mixer_callback(gcb,231,1,'QT')
      mask TypeOptions t231_QT_dac1_coarse_freq: 0
      mask TypeOptions t231_QT_dac1_nyquist_zone: Zone 1 | Zone 2
      mask TypeOptions t231_QT_dac1_decode_mode: SNR Optimized | Linearity Optimized
      mask Callback t231_QT_dac2_enable: enable_dac_opt(gcb,231,2,'QT');
      mask TypeOptions t231_QT_dac2_analog_output: Real | I/Q
      mask Callback t231_QT_dac2_analog_output:
      | validate_analog_data(gcb,231,2,'QT');
      | update_axis_clk(gcb,231);
      mask TypeOptions t231_QT_dac2_inter_mode: 1x | 2x | 3x | 4x | 5x | 6x | 8x | 10x | 12x | 16x | 20x | 24x | 40x
      mask Callback t231_QT_dac2_inter_mode:
      | % if I/Q output mode, need to copy interp factor before updating axis clk
      | % note only the even slice for the tile makes this check
      | if chk_param(gcb, 't231_QT_dac2_analog_output', 'I/Q')
      |   inter_mode = get_param(gcb, 't231_QT_dac2_inter_mode');
      |   set_param(gcb, 't231_QT_dac3_inter_mode', inter_mode);
      | end
      | update_axis_clk(gcb,231);
      mask TypeOptions t231_QT_dac2_sample_per_cycle: 4 | 5 | 6 | 7 | 8 | 9 | 10 | 11 | 12 | 13 | 14 | 15 | 16
      mask Callback t231_QT_dac2_sample_per_cycle:
      | % if I/Q output mode, need to copy samples per clk before updating axis clk
      | % note only the even slice for the tile makes this check
      | if chk_param(gcb, 't231_QT_dac2_analog_output', 'I/Q')
      |   spc = get_param(gcb, 't231_QT_dac2_sample_per_cycle');
      |   set_param(gcb, 't231_QT_dac3_sample_per_cycle', spc);
      | end
      | update_axis_clk_label(gcb,231);
      mask TypeOptions t231_QT_dac2_datapath_mode: DUC 0 to Fs/2 | DUC 0 to Fs/4 | DUC Fs/4 to Fs/2 | No DUC 0 to Fs/2
      mask TypeOptions t231_QT_dac2_mixer_type: Fine | Coarse
      mask Callback t231_QT_dac2_mixer_type: mixertype_callback(gcb,231,2,'QT');
      mask TypeOptions t231_QT_dac2_mixer_mode: Real -> Real | I/Q -> Real
      mask Callback t231_QT_dac2_mixer_mode: mixer_callback(gcb,231,2,'QT')
      mask TypeOptions t231_QT_dac2_coarse_freq: 0
      mask TypeOptions t231_QT_dac2_nyquist_zone: Zone 1 | Zone 2
      mask TypeOptions t231_QT_dac2_decode_mode: SNR Optimized | Linearity Optimized
      mask Callback t231_QT_dac3_enable: enable_dac_opt(gcb,231,3,'QT');
      mask TypeOptions t231_QT_dac3_analog_output: Real | I/Q
      mask Callback t231_QT_dac3_analog_output:
      | validate_analog_data(gcb,231,3,'QT');
      | update_axis_clk(gcb,231);
      mask TypeOptions t231_QT_dac3_inter_mode: 1x | 2x | 3x | 4x | 5x | 6x | 8x | 10x | 12x | 16x | 20x | 24x | 40x
      mask Callback t231_QT_dac3_inter_mode: update_axis_clk(gcb,231);
      mask TypeOptions t231_QT_dac3_sample_per_cycle: 4 | 5 | 6 | 7 | 8 | 9 | 10 | 11 | 12 | 13 | 14 | 15 | 16
      mask Callback t231_QT_dac3_sample_per_cycle: update_axis_clk_label(gcb,231);
      mask TypeOptions t231_QT_dac3_datapath_mode: DUC 0 to Fs/2 | DUC 0 to Fs/4 | DUC Fs/4 to Fs/2 | No DUC 0 to Fs/2
      mask TypeOptions t231_QT_dac3_mixer_type: Fine | Coarse
      mask Callback t231_QT_dac3_mixer_type: mixertype_callback(gcb,231,3,'QT');
      mask TypeOptions t231_QT_dac3_mixer_mode: Real -> Real | I/Q -> Real
      mask Callback t231_QT_dac3_mixer_mode: mixer_callback(gcb,231,3,'QT')
      mask TypeOptions t231_QT_dac3_coarse_freq: 0
      mask TypeOptions t231_QT_dac3_nyquist_zone: Zone 1 | Zone 2
      mask TypeOptions t231_QT_dac3_decode_mode: SNR Optimized | Linearity Optimized
      mask Callback t231_DT_dac0_enable: enable_dac_opt(gcb,231,0,'DT');
      mask TypeOptions t231_DT_dac0_analog_output: Real | I/Q
      mask Callback t231_DT_dac0_analog_output:
      | validate_analog_data(gcb,231,0,'DT');
      | update_axis_clk(gcb,231);
      mask TypeOptions t231_DT_dac0_inter_mode: 1x | 2x | 3x | 4x | 5x | 6x | 8x | 10x | 12x | 16x | 20x | 24x | 40x
      mask Callback t231_DT_dac0_inter_mode:
      | % if I/Q output mode, need to copy interp factor before updating axis clk
      | % note only the even slice for the tile makes this check
      | if chk_param(gcb, 't231_DT_dac0_analog_output', 'I/Q')
      |   inter_mode = get_param(gcb, 't231_DT_dac0_inter_mode');
      |   set_param(gcb, 't231_DT_dac1_inter_mode', inter_mode);
      | end
      | update_axis_clk(gcb,231);
      mask TypeOptions t231_DT_dac0_sample_per_cycle: 4 | 5 | 6 | 7 | 8 | 9 | 10 | 11 | 12 | 13 | 14 | 15 | 16
      mask Callback t231_DT_dac0_sample_per_cycle:
      | % if I/Q output mode, need to copy samples per clk before updating axis clk
      | % note only the even slice for the tile makes this check
      | if chk_param(gcb, 't231_DT_dac0_analog_output', 'I/Q')
      |   spc = get_param(gcb, 't231_DT_dac0_sample_per_cycle');
      |   set_param(gcb, 't231_DT_dac1_sample_per_cycle', spc);
      | end
      | update_axis_clk_label(gcb,231);
      mask TypeOptions t231_DT_dac0_mixer_type: Fine | Coarse
      mask Callback t231_DT_dac0_mixer_type: mixertype_callback(gcb,231,0,'DT');
      mask TypeOptions t231_DT_dac0_mixer_mode: Real -> Real | I/Q -> Real
      mask Callback t231_DT_dac0_mixer_mode: mixer_callback(gcb,231,0,'DT');
      mask TypeOptions t231_DT_dac0_coarse_freq: 0
      mask TypeOptions t231_DT_dac0_nyquist_zone: Zone 1 | Zone 2
      mask TypeOptions t231_DT_dac0_decode_mode: SNR Optimized | Linearity Optimized
      mask Callback t231_DT_dac1_enable: enable_dac_opt(gcb,231,1,'DT');
      mask TypeOptions t231_DT_dac1_analog_output: Real
      mask Callback t231_DT_dac1_analog_output:
      | validate_analog_data(gcb,231,1,'DT');
      | update_axis_clk(gcb,231);
      mask TypeOptions t231_DT_dac1_inter_mode: 1x | 2x | 3x | 4x | 5x | 6x | 8x | 10x | 12x | 16x | 20x | 24x | 40x
      mask Callback t231_DT_dac1_inter_mode: update_axis_clk(gcb,231);
      mask TypeOptions t231_DT_dac1_sample_per_cycle: 4 | 5 | 6 | 7 | 8 | 9 | 10 | 11 | 12 | 13 | 14 | 15 | 16
      mask Callback t231_DT_dac1_sample_per_cycle: update_axis_clk_label(gcb,231);
      mask TypeOptions t231_DT_dac1_mixer_type: Fine | Coarse
      mask Callback t231_DT_dac1_mixer_type: mixertype_callback(gcb,231,1,'DT');
      mask TypeOptions t231_DT_dac1_mixer_mode: Real -> Real | I/Q -> Real
      mask Callback t231_DT_dac1_mixer_mode: mixer_callback(gcb,231,1,'DT');
      mask TypeOptions t231_DT_dac1_coarse_freq: 0
      mask TypeOptions t231_DT_dac1_nyquist_zone: Zone 1 | Zone 2
      mask TypeOptions t231_DT_dac1_decode_mode: SNR Optimized | Linearity Optimized
      mask TypeOptions t224_adc_clk_src: 224 | 225 | 226 | 227 | 228 | 229 | 230 | 231
      mask TypeOptions t224_clk_dist: None | Input Refclk | PLL Output
      mask TypeOptions t225_adc_clk_src: 224 | 225 | 226 | 227 | 228 | 229 | 230 | 231
      mask TypeOptions t225_clk_dist: None | Input Refclk | PLL Output
      mask TypeOptions t226_adc_clk_src: 224 | 225 | 226 | 227 | 228 | 229 | 230 | 231
      mask TypeOptions t226_clk_dist: None | Input Refclk | PLL Output
      mask TypeOptions t227_adc_clk_src: 224 | 225 | 226 | 227 | 228 | 229 | 230 | 231
      mask TypeOptions t227_clk_dist: None | Input Refclk | PLL Output
      mask TypeOptions t228_dac_clk_src: 224 | 225 | 226 | 227 | 228 | 229 | 230 | 231
      mask TypeOptions t228_clk_dist: None | Input Refclk | PLL Output
      mask TypeOptions t229_dac_clk_src: 224 | 225 | 226 | 227 | 228 | 229 | 230 | 231
      mask TypeOptions t229_clk_dist: None | Input Refclk | PLL Output
      mask TypeOptions t230_dac_clk_src: 224 | 225 | 226 | 227 | 228 | 229 | 230 | 231
      mask TypeOptions t230_clk_dist: None | Input Refclk | PLL Output
      mask TypeOptions t231_dac_clk_src: 224 | 225 | 226 | 227 | 228 | 229 | 230 | 231
      mask TypeOptions t231_clk_dist: None | Input Refclk | PLL Output
      mask Callback maskdoneopening:
      | %assignin('base','mask_opening',0)
      | %assignin('base','run_init',1)
      | set_param(gcb,'maskopening','0')
      | set_param(gcb,'runinit','1')
      mask DialogControl ADCTileSelect Prompt: ADC Tiles
      mask DialogControl Tile224_container Prompt: Tile 224
      mask DialogControl pll_clocking_config_224 Prompt: Clocking and PLL Configuration
      mask DialogControl t224_QuadTileConfig Prompt: Quad Tile Configuration
      mask DialogControl t224_ADCPair01 Prompt: ADC Pair 0,1
      mask DialogControl t224_QT_adc0 Prompt: ADC 0
      mask DialogControl t224_QT_adc0_DataSettings Prompt: Data Settings
      mask DialogControl t224_QT_adc0_req_axis_clk_label Prompt: Required AXI4-Stream clock:
      mask DialogControl t224_QT_adc0_MixerSettings Prompt: MIxer Settings
      mask DialogControl t224_QT_adc0_AnalogSettings Prompt: Analog Settings
      mask DialogControl t224_QT_adc1 Prompt: ADC 1
      mask DialogControl t224_QT_adc1_DataSettings Prompt: Data Settings
      mask DialogControl t224_QT_adc1_req_axis_clk_label Prompt: Required AXI4-Stream clock:
      mask DialogControl t224_QT_adc1_MixerSettings Prompt: MIxer Settings
      mask DialogControl t224_QT_adc1_AnalogSettings Prompt: Analog Settings
      mask DialogControl ADCPair23 Prompt: ADC Pair 2,3
      mask DialogControl QT_adc2 Prompt: ADC 2
      mask DialogControl t224_QT_adc2_DataSettings Prompt: Data Settings
      mask DialogControl t224_QT_adc2_req_axis_clk_label Prompt: Required AXI4-Stream clock:
      mask DialogControl t224_QT_adc2_MixerSettings Prompt: MIxer Settings
      mask DialogControl t224_QT_adc2_AnalogSettings Prompt: Analog Settings
      mask DialogControl t224_QT_adc3 Prompt: ADC 3
      mask DialogControl t224_QT_adc3_DataSettings Prompt: Data Settings
      mask DialogControl t224_QT_adc3_req_axis_clk_label Prompt: Required AXI4-Stream clock:
      mask DialogControl t224_QT_adc3_MixerSettings Prompt: MIxer Settings
      mask DialogControl t224_QT_adc3_AnalogSettings Prompt: Analog Settings
      mask DialogControl t224_DualTileConfig Prompt: Dual Tile Configuration
      mask DialogControl t224_DT_adc0 Prompt: ADC 0
      mask DialogControl t224_DT_adc0_DataSettings Prompt: Data Settings
      mask DialogControl t224_DT_adc0_req_axis_clk_label Prompt: Required AXI4-Stream clock:
      mask DialogControl t224_DT_adc0_MixerSettings Prompt: MIxer Settings
      mask DialogControl t224_DT_adc0_AnalogSettings Prompt: Analog Settings
      mask DialogControl t224_DT_adc1 Prompt: ADC 1
      mask DialogControl t224_DT_adc1_DataSettings Prompt: Data Settings
      mask DialogControl t224_DT_adc1_req_axis_clk_label Prompt: Required AXI4-Stream clock:
      mask DialogControl t224_DT_adc1_MixerSettings Prompt: MIxer Settings
      mask DialogControl t224_DT_adc1_AnalogSettings Prompt: Analog Settings
      mask DialogControl Tile225_container Prompt: Tile 225
      mask DialogControl pll_clocking_config_225 Prompt: Clocking and PLL Configuration
      mask DialogControl t225_QuadTileConfig Prompt: Quad Tile Configuration
      mask DialogControl t225_ADCPair01 Prompt: ADC Pair 0,1
      mask DialogControl t225_QT_adc0 Prompt: ADC 0
      mask DialogControl t225_QT_adc0_DataSettings Prompt: Data Settings
      mask DialogControl t225_QT_adc0_req_axis_clk_label Prompt: Required AXI4-Stream clock:
      mask DialogControl t225_QT_adc0_MixerSettings Prompt: MIxer Settings
      mask DialogControl t225_QT_adc0_AnalogSettings Prompt: Analog Settings
      mask DialogControl t225_QT_adc1 Prompt: ADC 1
      mask DialogControl t225_QT_adc1_DataSettings Prompt: Data Settings
      mask DialogControl t225_QT_adc1_req_axis_clk_label Prompt: Required AXI4-Stream clock:
      mask DialogControl t225_QT_adc1_MixerSettings Prompt: MIxer Settings
      mask DialogControl t225_QT_adc1_AnalogSettings Prompt: Analog Settings
      mask DialogControl t225_ADCPair23 Prompt: ADC Pair 2,3
      mask DialogControl t225_QT_adc2 Prompt: ADC 2
      mask DialogControl t225_QT_adc2_DataSettings Prompt: Data Settings
      mask DialogControl t225_QT_adc2_req_axis_clk_label Prompt: Required AXI4-Stream clock:
      mask DialogControl t225_QT_adc2_MixerSettings Prompt: MIxer Settings
      mask DialogControl t225_QT_adc2_AnalogSettings Prompt: Analog Settings
      mask DialogControl t225_QT_adc3 Prompt: ADC 3
      mask DialogControl t225_QT_adc3_DataSettings Prompt: Data Settings
      mask DialogControl t225_QT_adc3_req_axis_clk_label Prompt: Required AXI4-Stream clock:
      mask DialogControl t225_QT_adc3_MixerSettings Prompt: MIxer Settings
      mask DialogControl t225_QT_adc3_AnalogSettings Prompt: Analog Settings
      mask DialogControl t225_DualTileConfig Prompt: Dual Tile Configuration
      mask DialogControl t225_DT_adc0 Prompt: ADC 0
      mask DialogControl t225_DT_adc0_DataSettings Prompt: Data Settings
      mask DialogControl t225_DT_adc0_req_axis_clk_label Prompt: Required AXI4-Stream clock:
      mask DialogControl t225_DT_adc0_MixerSettings Prompt: MIxer Settings
      mask DialogControl t225_DT_adc0_AnalogSettings Prompt: Analog Settings
      mask DialogControl t225_DT_adc1 Prompt: ADC 1
      mask DialogControl t225_DT_adc1_DataSettings Prompt: Data Settings
      mask DialogControl t225_DT_adc1_req_axis_clk_label Prompt: Required AXI4-Stream clock:
      mask DialogControl t225_DT_adc1_MixerSettings Prompt: MIxer Settings
      mask DialogControl t225_DT_adc1_AnalogSettings Prompt: Analog Settings
      mask DialogControl Tile226_container Prompt: Tile 226
      mask DialogControl pll_clocking_config_226 Prompt: Clocking and PLL Configuration
      mask DialogControl t226_QuadTileConfig Prompt: Quad Tile Configuration
      mask DialogControl t226_ADCPair01 Prompt: ADC Pair 0,1
      mask DialogControl t226_QT_adc0 Prompt: ADC 0
      mask DialogControl t226_QT_adc0_DataSettings Prompt: Data Settings
      mask DialogControl t226_QT_adc0_req_axis_clk_label Prompt: Required AXI4-Stream clock:
      mask DialogControl t226_QT_adc0_MixerSettings Prompt: MIxer Settings
      mask DialogControl t226_QT_adc0_AnalogSettings Prompt: Analog Settings
      mask DialogControl t226_QT_adc1 Prompt: ADC 1
      mask DialogControl t226_QT_adc1_DataSettings Prompt: Data Settings
      mask DialogControl t226_QT_adc1_req_axis_clk_label Prompt: Required AXI4-Stream clock:
      mask DialogControl t226_QT_adc1_MixerSettings Prompt: MIxer Settings
      mask DialogControl t226_QT_adc1_AnalogSettings Prompt: Analog Settings
      mask DialogControl t226_ADCPair23 Prompt: ADC Pair 2,3
      mask DialogControl t226_QT_adc2 Prompt: ADC 2
      mask DialogControl t226_QT_adc2_DataSettings Prompt: Data Settings
      mask DialogControl t226_QT_adc2_req_axis_clk_label Prompt: Required AXI4-Stream clock:
      mask DialogControl t226_QT_adc2_MixerSettings Prompt: MIxer Settings
      mask DialogControl t226_QT_adc2_AnalogSettings Prompt: Analog Settings
      mask DialogControl t226_QT_adc3 Prompt: ADC 3
      mask DialogControl t226_QT_adc3_DataSettings Prompt: Data Settings
      mask DialogControl t226_QT_adc3_req_axis_clk_label Prompt: Required AXI4-Stream clock:
      mask DialogControl t226_QT_adc3_MixerSettings Prompt: MIxer Settings
      mask DialogControl t226_QT_adc3_AnalogSettings Prompt: Analog Settings
      mask DialogControl t226_DualTileConfig Prompt: Dual Tile Configuration
      mask DialogControl t226_DT_adc0 Prompt: ADC 0
      mask DialogControl t226_DT_adc0_DataSettings Prompt: Data Settings
      mask DialogControl t226_DT_adc0_req_axis_clk_label Prompt: Required AXI4-Stream clock:
      mask DialogControl t226_DT_adc0_MixerSettings Prompt: MIxer Settings
      mask DialogControl t226_DT_adc0_AnalogSettings Prompt: Analog Settings
      mask DialogControl t226_DT_adc1 Prompt: ADC 1
      mask DialogControl t226_DT_adc1_DataSettings Prompt: Data Settings
      mask DialogControl t226_DT_adc1_req_axis_clk_label Prompt: Required AXI4-Stream clock:
      mask DialogControl t226_DT_adc1_MixerSettings Prompt: MIxer Settings
      mask DialogControl t226_DT_adc1_AnalogSettings Prompt: Analog Settings
      mask DialogControl Tile227_container Prompt: Tile 227
      mask DialogControl pll_clocking_config_227 Prompt: Clocking and PLL Configuration
      mask DialogControl t227_QuadTileConfig Prompt: Quad Tile Configuration
      mask DialogControl t227_ADCPair01 Prompt: ADC Pair 0,1
      mask DialogControl t227_QT_adc0 Prompt: ADC 0
      mask DialogControl t227_QT_adc0_DataSettings Prompt: Data Settings
      mask DialogControl t227_QT_adc0_req_axis_clk_label Prompt: Required AXI4-Stream clock:
      mask DialogControl t227_QT_adc0_MixerSettings Prompt: MIxer Settings
      mask DialogControl t227_QT_adc0_AnalogSettings Prompt: Analog Settings
      mask DialogControl t227_QT_adc1 Prompt: ADC 1
      mask DialogControl t227_QT_adc1_DataSettings Prompt: Data Settings
      mask DialogControl t227_QT_adc1_req_axis_clk_label Prompt: Required AXI4-Stream clock:
      mask DialogControl t227_QT_adc1_MixerSettings Prompt: MIxer Settings
      mask DialogControl t227_QT_adc1_AnalogSettings Prompt: Analog Settings
      mask DialogControl t227_ADCPair23 Prompt: ADC Pair 2,3
      mask DialogControl t227_QT_adc2 Prompt: ADC 2
      mask DialogControl t227_QT_adc2_DataSettings Prompt: Data Settings
      mask DialogControl t227_QT_adc2_req_axis_clk_label Prompt: Required AXI4-Stream clock:
      mask DialogControl t227_QT_adc2_MixerSettings Prompt: MIxer Settings
      mask DialogControl t227_QT_adc2_AnalogSettings Prompt: Analog Settings
      mask DialogControl t227_QT_adc3 Prompt: ADC 3
      mask DialogControl t227_QT_adc3_DataSettings Prompt: Data Settings
      mask DialogControl t227_QT_adc3_req_axis_clk_label Prompt: Required AXI4-Stream clock:
      mask DialogControl t227_QT_adc3_MixerSettings Prompt: MIxer Settings
      mask DialogControl t227_QT_adc3_AnalogSettings Prompt: Analog Settings
      mask DialogControl t227_DualTileConfig Prompt: Dual Tile Configuration
      mask DialogControl t227_DT_adc0 Prompt: ADC 0
      mask DialogControl t227_DT_adc0_DataSettings Prompt: Data Settings
      mask DialogControl t227_DT_adc0_req_axis_clk_label Prompt: Required AXI4-Stream clock:
      mask DialogControl t227_DT_adc0_MixerSettings Prompt: MIxer Settings
      mask DialogControl t227_DT_adc0_AnalogSettings Prompt: Analog Settings
      mask DialogControl t227_DT_adc1 Prompt: ADC 1
      mask DialogControl t227_DT_adc1_DataSettings Prompt: Data Settings
      mask DialogControl t227_DT_adc1_req_axis_clk_label Prompt: Required AXI4-Stream clock:
      mask DialogControl t227_DT_adc1_MixerSettings Prompt: MIxer Settings
      mask DialogControl t227_DT_adc1_AnalogSettings Prompt: Analog Settings
      mask DialogControl DACTileSelect Prompt: DAC Tiles
      mask DialogControl Tile228_container Prompt: Tile 228
      mask DialogControl pll_clocking_config_228 Prompt: Clocking and PLL Configuration
      mask DialogControl t228_QuadTileConfig Prompt: Quad Tile Configuration
      mask DialogControl t228_DACPair01 Prompt: DAC Pair 0,1
      mask DialogControl t228_QT_dac0 Prompt: DAC 0
      mask DialogControl t228_QT_dac0_DataSettings Prompt: Data Settings
      mask DialogControl t228_QT_dac0_req_axis_clk_label Prompt: Required AXI4-Stream clock:
      mask DialogControl t228_QT_dac0_MixerSettings Prompt: MIxer Settings
      mask DialogControl t228_QT_dac0_AnalogSettings Prompt: Analog Settings
      mask DialogControl t228_QT_dac1 Prompt: DAC 1
      mask DialogControl t228_QT_dac1_DataSettings Prompt: Data Settings
      mask DialogControl t228_QT_dac1_req_axis_clk_label Prompt: Required AXI4-Stream clock:
      mask DialogControl t228_QT_dac1_MixerSettings Prompt: MIxer Settings
      mask DialogControl t228_QT_dac1_AnalogSettings Prompt: Analog Settings
      mask DialogControl t228_DACPair23 Prompt: DAC Pair 2,3
      mask DialogControl t228_QT_dac2 Prompt: DAC 2
      mask DialogControl t228_QT_dac2_DataSettings Prompt: Data Settings
      mask DialogControl t228_QT_dac2_req_axis_clk_label Prompt: Required AXI4-Stream clock:
      mask DialogControl t228_QT_dac2_MixerSettings Prompt: MIxer Settings
      mask DialogControl t228_QT_dac2_AnalogSettings Prompt: Analog Settings
      mask DialogControl t228_QT_dac3 Prompt: DAC 3
      mask DialogControl t228_QT_dac3_DataSettings Prompt: Data Settings
      mask DialogControl t228_QT_dac3_req_axis_clk_label Prompt: Required AXI4-Stream clock:
      mask DialogControl t228_QT_dac3_MixerSettings Prompt: MIxer Settings
      mask DialogControl t228_QT_dac3_AnalogSettings Prompt: Analog Settings
      mask DialogControl t228_DualTileConfig Prompt: Dual Tile Configuration
      mask DialogControl t228_DT_dac0 Prompt: DAC 0
      mask DialogControl t228_DT_dac0_DataSettings Prompt: Data Settings
      mask DialogControl t228_DT_dac0_req_axis_clk_label Prompt: Required AXI4-Stream clock:
      mask DialogControl t228_DT_dac0_MixerSettings Prompt: MIxer Settings
      mask DialogControl t228_DT_dac0_AnalogSettings Prompt: Analog Settings
      mask DialogControl t228_DT_dac1 Prompt: DAC 1
      mask DialogControl t228_DT_dac1_DataSettings Prompt: Data Settings
      mask DialogControl t228_DT_dac1_req_axis_clk_label Prompt: Required AXI4-Stream clock:
      mask DialogControl t228_DT_dac1_MixerSettings Prompt: MIxer Settings
      mask DialogControl t228_DT_dac1_AnalogSettings Prompt: Analog Settings
      mask DialogControl Tile229_container Prompt: Tile 229
      mask DialogControl pll_clocking_config_229 Prompt: Clocking and PLL Configuration
      mask DialogControl t229_QuadTileConfig Prompt: Quad Tile Configuration
      mask DialogControl t229_DACPair01 Prompt: DAC Pair 0,1
      mask DialogControl t229_QT_dac0 Prompt: DAC 0
      mask DialogControl t229_QT_dac0_DataSettings Prompt: Data Settings
      mask DialogControl t229_QT_dac0_req_axis_clk_label Prompt: Required AXI4-Stream clock:
      mask DialogControl t229_QT_dac0_MixerSettings Prompt: MIxer Settings
      mask DialogControl t229_QT_dac0_AnalogSettings Prompt: Analog Settings
      mask DialogControl t229_QT_dac1 Prompt: DAC 1
      mask DialogControl t229_QT_dac1_DataSettings Prompt: Data Settings
      mask DialogControl t229_QT_dac1_req_axis_clk_label Prompt: Required AXI4-Stream clock:
      mask DialogControl t229_QT_dac1_MixerSettings Prompt: MIxer Settings
      mask DialogControl t229_QT_dac1_AnalogSettings Prompt: Analog Settings
      mask DialogControl t229_DACPair23 Prompt: DAC Pair 2,3
      mask DialogControl t229_QT_dac2 Prompt: DAC 2
      mask DialogControl t229_QT_dac2_DataSettings Prompt: Data Settings
      mask DialogControl t229_QT_dac2_req_axis_clk_label Prompt: Required AXI4-Stream clock:
      mask DialogControl t229_QT_dac2_MixerSettings Prompt: MIxer Settings
      mask DialogControl t229_QT_dac2_AnalogSettings Prompt: Analog Settings
      mask DialogControl t229_QT_dac3 Prompt: DAC 3
      mask DialogControl t229_QT_dac3_DataSettings Prompt: Data Settings
      mask DialogControl t229_QT_dac3_req_axis_clk_label Prompt: Required AXI4-Stream clock:
      mask DialogControl t229_QT_dac3_MixerSettings Prompt: MIxer Settings
      mask DialogControl t229_QT_dac3_AnalogSettings Prompt: Analog Settings
      mask DialogControl t229_DualTileConfig Prompt: Dual Tile Configuration
      mask DialogControl t229_DT_dac0 Prompt: DAC 0
      mask DialogControl t229_DT_dac0_DataSettings Prompt: Data Settings
      mask DialogControl t229_DT_dac0_req_axis_clk_label Prompt: Required AXI4-Stream clock:
      mask DialogControl t229_DT_dac0_MixerSettings Prompt: MIxer Settings
      mask DialogControl t229_DT_dac0_AnalogSettings Prompt: Analog Settings
      mask DialogControl t229_DT_dac1 Prompt: DAC 1
      mask DialogControl t229_DT_dac1_DataSettings Prompt: Data Settings
      mask DialogControl t229_DT_dac1_req_axis_clk_label Prompt: Required AXI4-Stream clock:
      mask DialogControl t229_DT_dac1_MixerSettings Prompt: MIxer Settings
      mask DialogControl t229_DT_dac1_AnalogSettings Prompt: Analog Settings
      mask DialogControl Tile230_container Prompt: Tile 230
      mask DialogControl pll_clocking_config_230 Prompt: Clocking and PLL Configuration
      mask DialogControl t230_QuadTileConfig Prompt: Quad Tile Configuration
      mask DialogControl t230_DACPair01 Prompt: DAC Pair 0,1
      mask DialogControl t230_QT_dac0 Prompt: DAC 0
      mask DialogControl t230_QT_dac0_DataSettings Prompt: Data Settings
      mask DialogControl t230_QT_dac0_req_axis_clk_label Prompt: Required AXI4-Stream clock:
      mask DialogControl t230_QT_dac0_MixerSettings Prompt: MIxer Settings
      mask DialogControl t230_QT_dac0_AnalogSettings Prompt: Analog Settings
      mask DialogControl t230_QT_dac1 Prompt: DAC 1
      mask DialogControl t230_QT_dac1_DataSettings Prompt: Data Settings
      mask DialogControl t230_QT_dac1_req_axis_clk_label Prompt: Required AXI4-Stream clock:
      mask DialogControl t230_QT_dac1_MixerSettings Prompt: MIxer Settings
      mask DialogControl t230_QT_dac1_AnalogSettings Prompt: Analog Settings
      mask DialogControl t230_DACPair23 Prompt: DAC Pair 2,3
      mask DialogControl t230_QT_dac2 Prompt: DAC 2
      mask DialogControl t230_QT_dac2_DataSettings Prompt: Data Settings
      mask DialogControl t230_QT_dac2_req_axis_clk_label Prompt: Required AXI4-Stream clock:
      mask DialogControl t230_QT_dac2_MixerSettings Prompt: MIxer Settings
      mask DialogControl t230_QT_dac2_AnalogSettings Prompt: Analog Settings
      mask DialogControl t230_QT_dac3 Prompt: DAC 3
      mask DialogControl t230_QT_dac3_DataSettings Prompt: Data Settings
      mask DialogControl t230_QT_dac3_req_axis_clk_label Prompt: Required AXI4-Stream clock:
      mask DialogControl t230_QT_dac3_MixerSettings Prompt: MIxer Settings
      mask DialogControl t230_QT_dac3_AnalogSettings Prompt: Analog Settings
      mask DialogControl t230_DualTileConfig Prompt: Dual Tile Configuration
      mask DialogControl t230_DT_dac0 Prompt: DAC 0
      mask DialogControl t230_DT_dac0_DataSettings Prompt: Data Settings
      mask DialogControl t230_DT_dac0_req_axis_clk_label Prompt: Required AXI4-Stream clock:
      mask DialogControl t230_DT_dac0_MixerSettings Prompt: MIxer Settings
      mask DialogControl t230_DT_dac0_AnalogSettings Prompt: Analog Settings
      mask DialogControl t230_DT_dac1 Prompt: DAC 1
      mask DialogControl t230_DT_dac1_DataSettings Prompt: Data Settings
      mask DialogControl t230_DT_dac1_req_axis_clk_label Prompt: Required AXI4-Stream clock:
      mask DialogControl t230_DT_dac1_MixerSettings Prompt: MIxer Settings
      mask DialogControl t230_DT_dac1_AnalogSettings Prompt: Analog Settings
      mask DialogControl Tile231_container Prompt: Tile 231
      mask DialogControl pll_clocking_config_231 Prompt: Clocking and PLL Configuration
      mask DialogControl t231_QuadTileConfig Prompt: Quad Tile Configuration
      mask DialogControl t231_DACPair01 Prompt: DAC Pair 0,1
      mask DialogControl t231_QT_dac0 Prompt: DAC 0
      mask DialogControl t231_QT_dac0_DataSettings Prompt: Data Settings
      mask DialogControl t231_QT_dac0_req_axis_clk_label Prompt: Required AXI4-Stream clock:
      mask DialogControl t231_QT_dac0_MixerSettings Prompt: MIxer Settings
      mask DialogControl t231_QT_dac0_AnalogSettings Prompt: Analog Settings
      mask DialogControl t231_QT_dac1 Prompt: DAC 1
      mask DialogControl t231_QT_dac1_DataSettings Prompt: Data Settings
      mask DialogControl t231_QT_dac1_req_axis_clk_label Prompt: Required AXI4-Stream clock:
      mask DialogControl t231_QT_dac1_MixerSettings Prompt: MIxer Settings
      mask DialogControl t231_QT_dac1_AnalogSettings Prompt: Analog Settings
      mask DialogControl t231_DACPair23 Prompt: DAC Pair 2,3
      mask DialogControl t231_QT_dac2 Prompt: DAC 2
      mask DialogControl t231_QT_dac2_DataSettings Prompt: Data Settings
      mask DialogControl t231_QT_dac2_req_axis_clk_label Prompt: Required AXI4-Stream clock:
      mask DialogControl t231_QT_dac2_MixerSettings Prompt: MIxer Settings
      mask DialogControl t231_QT_dac2_AnalogSettings Prompt: Analog Settings
      mask DialogControl t231_QT_dac3 Prompt: DAC 3
      mask DialogControl t231_QT_dac3_DataSettings Prompt: Data Settings
      mask DialogControl t231_QT_dac3_req_axis_clk_label Prompt: Required AXI4-Stream clock:
      mask DialogControl t231_QT_dac3_MixerSettings Prompt: MIxer Settings
      mask DialogControl t231_QT_dac3_AnalogSettings Prompt: Analog Settings
      mask DialogControl t231_DualTileConfig Prompt: Dual Tile Configuration
      mask DialogControl t231_DT_dac0 Prompt: DAC 0
      mask DialogControl t231_DT_dac0_DataSettings Prompt: Data Settings
      mask DialogControl t231_DT_dac0_req_axis_clk_label Prompt: Required AXI4-Stream clock:
      mask DialogControl t231_DT_dac0_MixerSettings Prompt: MIxer Settings
      mask DialogControl t231_DT_dac0_AnalogSettings Prompt: Analog Settings
      mask DialogControl t231_DT_dac1 Prompt: DAC 1
      mask DialogControl t231_DT_dac1_DataSettings Prompt: Data Settings
      mask DialogControl t231_DT_dac1_req_axis_clk_label Prompt: Required AXI4-Stream clock:
      mask DialogControl t231_DT_dac1_MixerSettings Prompt: MIxer Settings
      mask DialogControl t231_DT_dac1_AnalogSettings Prompt: Analog Settings
      mask DialogControl SystemClocking Prompt: System Clocking
      mask DialogControl ADCClocking Prompt: ADC Tile Clocking
      mask DialogControl t224_clock_config Prompt: ADC Tile 224
      mask DialogControl t225_clock_config Prompt: ADC Tile 225
      mask DialogControl t226_clock_config Prompt: ADC Tile 226
      mask DialogControl t227_clock_config Prompt: ADC Tile 227
      mask DialogControl DACClocking Prompt: DAC Tile Clocking
      mask DialogControl t228_clock_config Prompt: DAC Tile 228
      mask DialogControl t229_clock_config Prompt: DAC Tile 229
      mask DialogControl t230_clock_config Prompt: DAC Tile 230
      mask DialogControl t231_clock_config Prompt: DAC Tile 231
  simple_bram_vacc1 : Subsystem  AncestorBlock=casper_library_accumulators/simple_bram_vacc  mask(simple_bram_vacc){vec_len=8192, arith_type=Unsigned, n_bits=64, bin_pt=34}
      mask prompts: vec_len "Vector length:"; arith_type "Output type:"; n_bits "Bit width (output):"; bin_pt "Binary point (output):"
      mask help: This simple vector accumulator is based on a shift register. It outputs its previous accumulated vector after a new_acc pulse is received.
      mask init:
      | simple_bram_vacc_init(gcb, ...
      |     'vec_len', vec_len, ...
      |     'arith_type', arith_type, ...
      |     'n_bits', n_bits, ...
      |     'bin_pt', bin_pt);
      mask TypeOptions arith_type: Signed | Unsigned
  simple_bram_vacc16 : Subsystem  AncestorBlock=casper_library_accumulators/simple_bram_vacc  mask(simple_bram_vacc){vec_len=8192, arith_type=Unsigned, n_bits=64, bin_pt=34}
      mask prompts: vec_len "Vector length:"; arith_type "Output type:"; n_bits "Bit width (output):"; bin_pt "Binary point (output):"
      mask help: This simple vector accumulator is based on a shift register. It outputs its previous accumulated vector after a new_acc pulse is received.
      mask init:
      | simple_bram_vacc_init(gcb, ...
      |     'vec_len', vec_len, ...
      |     'arith_type', arith_type, ...
      |     'n_bits', n_bits, ...
      |     'bin_pt', bin_pt);
      mask TypeOptions arith_type: Signed | Unsigned
  simple_bram_vacc2 : Subsystem  AncestorBlock=casper_library_accumulators/simple_bram_vacc  mask(simple_bram_vacc){vec_len=8192, arith_type=Unsigned, n_bits=64, bin_pt=34}
      mask prompts: vec_len "Vector length:"; arith_type "Output type:"; n_bits "Bit width (output):"; bin_pt "Binary point (output):"
      mask help: This simple vector accumulator is based on a shift register. It outputs its previous accumulated vector after a new_acc pulse is received.
      mask init:
      | simple_bram_vacc_init(gcb, ...
      |     'vec_len', vec_len, ...
      |     'arith_type', arith_type, ...
      |     'n_bits', n_bits, ...
      |     'bin_pt', bin_pt);
      mask TypeOptions arith_type: Signed | Unsigned
  simple_bram_vacc3 : Subsystem  AncestorBlock=casper_library_accumulators/simple_bram_vacc  mask(simple_bram_vacc){vec_len=8192, arith_type=Unsigned, n_bits=64, bin_pt=34}
      mask prompts: vec_len "Vector length:"; arith_type "Output type:"; n_bits "Bit width (output):"; bin_pt "Binary point (output):"
      mask help: This simple vector accumulator is based on a shift register. It outputs its previous accumulated vector after a new_acc pulse is received.
      mask init:
      | simple_bram_vacc_init(gcb, ...
      |     'vec_len', vec_len, ...
      |     'arith_type', arith_type, ...
      |     'n_bits', n_bits, ...
      |     'bin_pt', bin_pt);
      mask TypeOptions arith_type: Signed | Unsigned
  simple_bram_vacc4 : Subsystem  AncestorBlock=casper_library_accumulators/simple_bram_vacc  mask(simple_bram_vacc){vec_len=8192, arith_type=Unsigned, n_bits=64, bin_pt=34}
      mask prompts: vec_len "Vector length:"; arith_type "Output type:"; n_bits "Bit width (output):"; bin_pt "Binary point (output):"
      mask help: This simple vector accumulator is based on a shift register. It outputs its previous accumulated vector after a new_acc pulse is received.
      mask init:
      | simple_bram_vacc_init(gcb, ...
      |     'vec_len', vec_len, ...
      |     'arith_type', arith_type, ...
      |     'n_bits', n_bits, ...
      |     'bin_pt', bin_pt);
      mask TypeOptions arith_type: Signed | Unsigned
  simple_bram_vacc5 : Subsystem  AncestorBlock=casper_library_accumulators/simple_bram_vacc  mask(simple_bram_vacc){vec_len=8192, arith_type=Unsigned, n_bits=64, bin_pt=34}
      mask prompts: vec_len "Vector length:"; arith_type "Output type:"; n_bits "Bit width (output):"; bin_pt "Binary point (output):"
      mask help: This simple vector accumulator is based on a shift register. It outputs its previous accumulated vector after a new_acc pulse is received.
      mask init:
      | simple_bram_vacc_init(gcb, ...
      |     'vec_len', vec_len, ...
      |     'arith_type', arith_type, ...
      |     'n_bits', n_bits, ...
      |     'bin_pt', bin_pt);
      mask TypeOptions arith_type: Signed | Unsigned
  simple_bram_vacc6 : Subsystem  AncestorBlock=casper_library_accumulators/simple_bram_vacc  mask(simple_bram_vacc){vec_len=8192, arith_type=Unsigned, n_bits=64, bin_pt=34}
      mask prompts: vec_len "Vector length:"; arith_type "Output type:"; n_bits "Bit width (output):"; bin_pt "Binary point (output):"
      mask help: This simple vector accumulator is based on a shift register. It outputs its previous accumulated vector after a new_acc pulse is received.
      mask init:
      | simple_bram_vacc_init(gcb, ...
      |     'vec_len', vec_len, ...
      |     'arith_type', arith_type, ...
      |     'n_bits', n_bits, ...
      |     'bin_pt', bin_pt);
      mask TypeOptions arith_type: Signed | Unsigned
  simple_bram_vacc7 : Subsystem  AncestorBlock=casper_library_accumulators/simple_bram_vacc  mask(simple_bram_vacc){vec_len=8192, arith_type=Unsigned, n_bits=64, bin_pt=34}
      mask prompts: vec_len "Vector length:"; arith_type "Output type:"; n_bits "Bit width (output):"; bin_pt "Binary point (output):"
      mask help: This simple vector accumulator is based on a shift register. It outputs its previous accumulated vector after a new_acc pulse is received.
      mask init:
      | simple_bram_vacc_init(gcb, ...
      |     'vec_len', vec_len, ...
      |     'arith_type', arith_type, ...
      |     'n_bits', n_bits, ...
      |     'bin_pt', bin_pt);
      mask TypeOptions arith_type: Signed | Unsigned
  spect_cnt1 : xbsIndex_r4/Counter  cnt_type=Free Running  cnt_to=Inf  operation=Up  start_count=0  cnt_by_val=1  arith_type=Unsigned  n_bits=13  bin_pt=0  load_pin=off  rst=on  en=on  explicit_period=on  period=1  use_behavioral_HDL=off  implementation=Fabric  use_rpm=off  dbl_ovrd=off  block_type=counter
  sync_cnt : Subsystem  Tag=xps:sw_reg  AncestorBlock=xps_library/Memory/software_register  mask(swreg){io_dir=To Processor, io_delay=0, init_val=0, sample_period=1, names=reg, bitwidths=32, bin_pts=0, arith_types=0, sim_port=on, show_format=off}
      mask prompts: io_dir "I/O direction"; io_delay "I/O delay"; init_val "Initial Value"; sample_period "Sample period"; names "Bitfield names [msb...lsb]"; bitwidths "Bitfield widths"; bin_pts "Bitfield binary pts"; arith_types "Bitfield types, ufix=0, fix=1, bool=2"; sim_port "Provide sim input/output?"; show_format "Print format string?"
      mask help: A 32-bit software-accessible register. Can be divided into bitfields of varying widths and types using the fields in the block mask.
      mask init:
      | swreg_init(gcb)
      settings: AttributesFormatString=1output
      mask TypeOptions io_dir: To Processor | From Processor
      mask Callback io_dir:
      | mask_enables = get_param(gcb, 'MaskEnables');
      | mask_names = get_param(gcb, 'MaskNames');
      | if strcmp(get_param(gcb, 'io_dir'), 'To Processor'),
      |     mask_enables{ismember(mask_names, 'sample_period')} = 'off';
      | else
      |     mask_enables{ismember(mask_names, 'sample_period')} = 'on';
      | end
      | set_param(gcb, 'MaskEnables', mask_enables);
      mask DialogControl ParameterTabVar0 Prompt: Setup
  sync_cntr : xbsIndex_r4/Counter  cnt_type=Free Running  cnt_to=Inf  operation=Up  start_count=0  cnt_by_val=1  arith_type=Unsigned  n_bits=32  bin_pt=0  load_pin=off  rst=on  en=on  explicit_period=on  period=1  use_behavioral_HDL=off  implementation=Fabric  use_rpm=off  dbl_ovrd=off  block_type=counter
  sync_gen : Subsystem  AncestorBlock=casper_library_misc/sync_gen  mask(sync_gen){sim_acc_len=1, fft_size=256, fft_simult_inputs=16, pfb_fir_taps=8, reorder_vec=[2  2  4], scale=256}
      mask prompts: sim_acc_len "Simulation Accumulation Length"; fft_size "FFT Size"; fft_simult_inputs "Simultaneous Inputs (FFT)"; pfb_fir_taps "Taps in pfb_fir (use 1 if no pfb_fir)"; reorder_vec "Reorder Orders (e.g. [2 2 2])"
      mask help:
      | This block computes the sync period based on system parameters as
      | described in Casper memo.  Detailed descritions of the block's
      | variables can be found in the 'Block Documentation' section of
      | the CASPER wiki.
      mask init:
      | sync_gen_init(gcb, ...
      |     'sim_acc_len', sim_acc_len, ...
      |     'fft_size', fft_size, ...
      |     'fft_simult_inputs', fft_simult_inputs,...
      |     'pfb_fir_taps', pfb_fir_taps, ...
      |     'reorder_vec', reorder_vec, ...
      |     'scale', scale);
      settings: AttributesFormatString=sim_sync_period=131072
      mask Help:
      | SyncPeriod=LCM(reorder_vec)*(acc_num)*(pfb_fir_len)*(fft_size/fft_simult_inputs)
      | 
      | See CASPER sync pulse memo for more details.
  wires:
  rfdc/3(m10_axis_tdata) -> Terminator1/1
  rfdc/2(m02_axis_tdata) -> Mux/3
  Mux/1 -> bus_expand1/1(bus_in)
  rfdc/8(m32_axis_tdata) -> Terminator3/1
  rfdc/5(m20_axis_tdata) -> Mux/4
  rfdc/7(m30_axis_tdata) -> Terminator2/1
  rfdc/4(m12_axis_tdata) -> Terminator11/1
  rfdc/6(m22_axis_tdata) -> Mux/5
  rfdc/1(m00_axis_tdata) -> Mux/2
  [adc_chan_sel] -> Mux/1
  Constant/1 -> adc_chan_sel/1(sim_1)
  adc_chan_sel/1(in_reg) -> [adc_chan_sel]
  sync_gen/1(sync_out) -> Delay33/1
  Delay33/1 -> [sync_gen]
  Constant3/1 -> acc_len/1(sim_1)
  [cnt_rst] -> acc_cntr/1
  acc_len/1(in_reg) -> pipeline2/1(d)
  Delay23/1 -> acc_cntr/2
  Delay6/1 -> acc_cnt/1(out_reg)
  sync_cntr/1 -> Delay21/1
  Delay21/1 -> sync_cnt/1(out_reg)
  acc_cnt/1(sim_out_reg) -> Terminator6/1
  acc_cntr/1 -> Delay6/1
  Constant2/1 -> cnt_rst/1(sim_1)
  pipeline2/1(q) -> [acc_len]
  [cnt_rst] -> sync_cntr/1
  cnt_rst/1(in_reg) -> pipeline1/1(d)
  [sync_gen] -> sync_cntr/2
  [new_acc] -> Delay23/1
  pipeline1/1(q) -> [cnt_rst]
  sync_cnt/1(sim_out_reg) -> Terminator7/1
  Counter25/1 -> Convert3/1
  Convert3/1 -> [en_ctrl2]
  [pfb1_sync] -> Counter25/1
  simple_bram_vacc16/2(valid) -> pipeline21/1(d)
  Reinterpret1/1 -> pipeline34/1(d)
  pipeline24/1(q) -> q10/2(data_in)
  pipeline70/1(q) -> pipeline6/1(d)
  simple_bram_vacc3/2(valid) -> pipeline49/1(d)
  simple_bram_vacc1/1(dout) -> Reinterpret9/1
  simple_bram_vacc7/2(valid) -> spect_cnt1/2, pipeline18/1(d)
  simple_bram_vacc2/2(valid) -> pipeline28/1(d)
  Delay54/1 -> power4/1
  fft2/5(out03) -> Delay47/1
  [cnt_rst] -> acc_cntrl1/3(rst)
  [new_acc] -> pipeline13/1(d)
  pipeline30/1(q) -> q12/1(addr)
  [new_acc] -> pipeline5/1(d)
  pipeline12/1(q) -> pipeline17/1(d)
  pipeline22/1(q) -> q10/1(addr)
  fft2/6(out04) -> Delay52/1
  Reinterpret6/1 -> pipeline48/1(d)
  pipeline17/1(q) -> simple_bram_vacc16/2(din)
  pipeline13/1(q) -> spect_cnt1/1
  pipeline52/1(q) -> q16/3(we)
  Delay56/1 -> pipeline47/1(d)
  Delay34/1 -> Delay32/1
  pipeline14/1(q) -> simple_bram_vacc7/1(new_acc)
  pipeline10/1(q) -> simple_bram_vacc3/2(din)
  Delay45/1 -> pipeline35/1(d)
  pipeline49/1(q) -> q15/3(we)
  [new_acc] -> pipeline36/1(d)
  q16/1(data_out) -> Terminator37/1
  Delay94/1 -> power7/1
  Reinterpret3/1 -> pipeline24/1(d)
  pipeline35/1(q) -> pipeline37/1(d)
  pipeline18/1(q) -> q9/3(we)
  Delay36/1 -> Delay37/1
  Delay39/1 -> acc_cntrl1/2(sync)
  [new_acc] -> pipeline42/1(d)
  pipeline11/1(q) -> q13/2(data_in)
  pipeline46/1(q) -> q14/1(addr)
  pipeline38/1(q) -> q9/2(data_in)
  pipeline59/1(q) -> q16/1(addr)
  fft2/1(sync_out) -> Delay34/1
  pipeline34/1(q) -> q12/2(data_in)
  Reinterpret9/1 -> pipeline27/1(d)
